simulink model "turbo_controller"  (R2025a)
settings: Solver=FixedStepAuto  StartTime=0.0  StopTime=inf  FixedStep=0.001  RelTol=1e-3
PostLoadFcn:
  | % 自动定位同目录CubeMX文件；不需要外部初始化脚本。
  | codertarget.data.setParameterValue('turbo_controller','STM32CubeMX.ProjectFile',fullfile(fileparts(get_param('turbo_controller','FileName')),'turbo_f407.ioc'));
InitFcn:
  | % 中文说明：按原控制器字段与类型创建三组接口总线；控制参数已内嵌。
  | tc_names=["EValve_Cycle" "EValve_Open" "Eblast_Cycle" "Eblast_Open" "Motor_Cycle" "Motor_Open" "EValve_Enable" "Eblast_Enable" "Motor_Enable" "SWO_Firework" "SWO_BleedAir" "EngineState" "Flag_ECUReset_Clear" "Flag_ECUReset_Save" "Flag_Reset_Enable" "Accelerator" "Nc_dem" "Nc"]; tc_types=["uint16" "uint16" "uint16" "uint16" "uint16" "uint16" "uint8" "uint8" "uint8" "uint8" "uint8" "uint8" "uint8" "uint8" "uint8" "single" "single" "single"];
  | for tc_k=1:numel(tc_names)
  |  tc_e(tc_k)=Simulink.BusElement; tc_e(tc_k).Name=char(tc_names(tc_k)); tc_e(tc_k).DataType=char(tc_types(tc_k));
  | end
  | EngineControl_Out=Simulink.Bus; EngineControl_Out.DataScope='Exported'; EngineControl_Out.Elements=tc_e;
  | clear tc_e tc_names tc_types tc_k
  | tc_names=["savedata1" "savedata2" "savedata3" "savedata4" "savedata5" "savedata6" "savedata7" "savedata8" "savedata9" "savedata10" "savedata11" "savedata12" "savedata13" "savedata14" "savedata15" "savedata16" "savedata17" "savedata18" "savedata19" "savedata20" "savedata21" "savedata22" "savedata23" "savedata24" "savedata25"]; tc_types=["single" "single" "single" "single" "single" "single" "single" "single" "single" "single" "single" "single" "single" "single" "single" "single" "single" "single" "single" "single" "single" "single" "single" "single" "single"];
  | for tc_k=1:numel(tc_names)
  |  tc_e(tc_k)=Simulink.BusElement; tc_e(tc_k).Name=char(tc_names(tc_k)); tc_e(tc_k).DataType=char(tc_types(tc_k));
  | end
  | SaveData_Out=Simulink.Bus; SaveData_Out.DataScope='Exported'; SaveData_Out.Elements=tc_e;
  | clear tc_e tc_names tc_types tc_k
  | tc_names=["senddata1" "senddata2" "senddata3" "senddata4" "senddata5" "senddata6" "senddata7" "senddata8" "senddata9" "senddata10" "senddata11" "senddata12" "senddata13" "senddata14" "senddata15" "senddata16" "senddata17" "senddata18" "senddata19" "senddata20" "senddata21" "senddata22" "senddata23" "senddata24" "senddata25" "senddata26" "senddata27" "senddata28" "senddata29"]; tc_types=["uint8" "uint8" "uint8" "uint8" "uint8" "uint8" "uint8" "uint8" "uint8" "uint8" "uint8" "uint8" "uint8" "uint8" "uint8" "uint8" "uint8" "uint8" "uint8" "uint8" "uint8" "uint8" "uint8" "uint8" "uint8" "uint8" "uint8" "uint8" "uint8"];
  | for tc_k=1:numel(tc_names)
  |  tc_e(tc_k)=Simulink.BusElement; tc_e(tc_k).Name=char(tc_names(tc_k)); tc_e(tc_k).DataType=char(tc_types(tc_k));
  | end
  | SendData_Out=Simulink.Bus; SendData_Out.DataScope='Exported'; SendData_Out.Elements=tc_e;
  | clear tc_e tc_names tc_types tc_k
  | 
  | % 以下为接口中文说明；只设置描述，不改变数值或数据类型。
  | EngineControl_Out.Description='执行控制输出（阀、电机、点火、状态及复位请求）';
  | tc_cn=["EValve_Cycle（主油阀周期计数（每计数2毫秒））" "EValve_Open（主油阀开通计数（每计数2毫秒））" "Eblast_Cycle（副油阀周期计数（每计数2毫秒））" "Eblast_Open（副油阀开通计数（每计数2毫秒））" "Motor_Cycle（起动电机周期计数）" "Motor_Open（起动电机开通计数）" "EValve_Enable（主油阀驱动使能）" "Eblast_Enable（副油阀驱动使能）" "Motor_Enable（起动电机使能）" "SWO_Firework（点火器使能（1开））" "SWO_BleedAir（引气阀使能（1开））" "EngineState（发动机状态）" "Flag_ECUReset_Clear（清除复位恢复状态请求）" "Flag_ECUReset_Save（保存复位恢复数据请求）" "Flag_Reset_Enable（处理器软件复位请求）" "Accelerator（油门／油泵给定控制量）" "Nc_dem（控制目标转速）" "Nc（发动机反馈转速（转每分））"];
  | tc_elements=EngineControl_Out.Elements;
  | for tc_k=1:numel(tc_cn)
  |  tc_elements(tc_k).Description=char(tc_cn(tc_k));
  | end
  | EngineControl_Out.Elements=tc_elements;
  | clear tc_cn tc_elements tc_k
  | SaveData_Out.Description='25项运行记录；字段含义按当前模型数据来源解释';
  | tc_cn=["savedata1（指令回显记录）" "savedata2（入口总温记录（℃））" "savedata3（电源电压记录）" "savedata4（排气温度记录（℃））" "savedata5（标定燃油压力记录）" "savedata6（副油阀占空比记录（％））" "savedata7（主油阀占空比记录（％））" "savedata8（温度修正转速记录）" "savedata9（开关输出及反馈位域）" "savedata10（物理转速记录）" "savedata11（油泵目标给定原始值）" "savedata12（起动电机占空比记录（％））" "savedata13（发动机状态码记录）" "savedata14（故障告警位域记录）" "savedata15（模型记录帧序号）" "savedata16（处理器温度记录（℃））" "savedata17（装订转速记录（沿用旧电源字段名））" "savedata18（导航高度记录）" "savedata19（飞行空速记录）" "savedata20（主阀旧记录位（恒零保留））" "savedata21（第21项保留记录（恒零））" "savedata22（保留记录项22）" "savedata23（保留记录项23）" "savedata24（保留记录项24）" "savedata25（保留记录项25）"];
  | tc_elements=SaveData_Out.Elements;
  | for tc_k=1:numel(tc_cn)
  |  tc_elements(tc_k).Description=char(tc_cn(tc_k));
  | end
  | SaveData_Out.Elements=tc_elements;
  | clear tc_cn tc_elements tc_k
  | SendData_Out.Description='29字段回传及外设命令接口；板端上位机帧只取第3至27字段';
  | tc_cn=["senddata1（回传发送允许标志（不直接上线路））" "senddata2（回传载荷长度25字节）" "senddata3（回传指令回显字节）" "senddata4（总温编码字节（℃＋80））" "senddata5（电源电压编码字节）" "senddata6（排温编码高字节）" "senddata7（排温编码低字节）" "senddata8（燃油压力编码高字节）" "senddata9（燃油压力编码低字节）" "senddata10（副油阀占空比字节（％））" "senddata11（主油阀占空比字节（％））" "senddata12（修正转速编码高字节）" "senddata13（修正转速编码低字节）" "senddata14（驱动及反馈状态位域）" "senddata15（物理转速编码高字节）" "senddata16（物理转速编码低字节）" "senddata17（油泵目标给定高字节（串口二使用））" "senddata18（油泵目标给定低字节（串口二使用））" "senddata19（起动电机占空比命令（串口一使用））" "senddata20（发动机状态码字节）" "senddata21（故障告警位域字节）" "senddata22（帧序号占位（板端另行填写））" "senddata23（处理器温度编码（℃＋50））" "senddata24（控制目标转速编码高字节）" "senddata25（控制目标转速编码低字节）" "senddata26（占位字节（板端改填实测泵速高字节））" "senddata27（占位字节（板端改填实测泵速低字节））" "senddata28（装订转速高字节（本板未发送））" "senddata29（装订转速低字节（本板未发送））"];
  | tc_elements=SendData_Out.Elements;
  | for tc_k=1:numel(tc_cn)
  |  tc_elements(tc_k).Description=char(tc_cn(tc_k));
  | end
  | SendData_Out.Elements=tc_elements;
  | clear tc_cn tc_elements tc_k
  | 
  | 
  | % FRAM模块化事务：接口类型和上电初始状态，随模型保存，无外部初始化文件。
  | clear FM_elements
  | FM_elements(1)=Simulink.BusElement;FM_elements(1).Name='phase';FM_elements(1).DataType='uint8';FM_elements(1).Dimensions=[1 1];FM_elements(1).Description='phase（当前事务阶段）';
  | FM_elements(2)=Simulink.BusElement;FM_elements(2).Name='a';FM_elements(2).DataType='uint8';FM_elements(2).Dimensions=[64 1];FM_elements(2).Description='a（启动时缓存的首区64字节）';
  | FM_elements(3)=Simulink.BusElement;FM_elements(3).Name='active';FM_elements(3).DataType='uint16';FM_elements(3).Dimensions=[1 1];FM_elements(3).Description='active（当前有效记录区地址）';
  | FM_elements(4)=Simulink.BusElement;FM_elements(4).Name='generation';FM_elements(4).DataType='uint32';FM_elements(4).Dimensions=[1 1];FM_elements(4).Description='generation（当前有效记录代号）';
  | FM_elements(5)=Simulink.BusElement;FM_elements(5).Name='record';FM_elements(5).DataType='uint8';FM_elements(5).Dimensions=[64 1];FM_elements(5).Description='record（本次冻结的待写记录）';
  | FM_elements(6)=Simulink.BusElement;FM_elements(6).Name='addr';FM_elements(6).DataType='uint16';FM_elements(6).Dimensions=[1 1];FM_elements(6).Description='addr（本次备用写入地址）';
  | FM_elements(7)=Simulink.BusElement;FM_elements(7).Name='lastSave';FM_elements(7).DataType='single';FM_elements(7).Dimensions=[1 1];FM_elements(7).Description='lastSave（上次开始保存的秒数）';
  | FM_elements(8)=Simulink.BusElement;FM_elements(8).Name='lastState';FM_elements(8).DataType='uint8';FM_elements(8).Dimensions=[1 1];FM_elements(8).Description='lastState（上次保存时的发动机状态）';
  | FM_elements(9)=Simulink.BusElement;FM_elements(9).Name='boot';FM_elements(9).DataType='boolean';FM_elements(9).Dimensions=[1 1];FM_elements(9).Description='boot（启动记录是否允许恢复）';
  | FM_elements(10)=Simulink.BusElement;FM_elements(10).Name='consumed';FM_elements(10).DataType='boolean';FM_elements(10).Dimensions=[1 1];FM_elements(10).Description='consumed（本次启动恢复通知是否已发送）';
  | FM_elements(11)=Simulink.BusElement;FM_elements(11).Name='payload';FM_elements(11).DataType='uint8';FM_elements(11).Dimensions=[20 1];FM_elements(11).Description='payload（当前20字节恢复内容）';
  | FM_elements(12)=Simulink.BusElement;FM_elements(12).Name='failures';FM_elements(12).DataType='uint32';FM_elements(12).Dimensions=[1 1];FM_elements(12).Description='failures（累计写后验证失败次数）';
  | FM_State=Simulink.Bus;FM_State.Elements=FM_elements;
  | clear FM_elements
  | FM_elements(1)=Simulink.BusElement;FM_elements(1).Name='validA';FM_elements(1).DataType='boolean';FM_elements(1).Dimensions=[1 1];FM_elements(1).Description='validA（首区记录有效）';
  | FM_elements(2)=Simulink.BusElement;FM_elements(2).Name='validB';FM_elements(2).DataType='boolean';FM_elements(2).Dimensions=[1 1];FM_elements(2).Description='validB（本次读回记录有效）';
  | FM_elements(3)=Simulink.BusElement;FM_elements(3).Name='generationA';FM_elements(3).DataType='uint32';FM_elements(3).Dimensions=[1 1];FM_elements(3).Description='generationA（首区代号）';
  | FM_elements(4)=Simulink.BusElement;FM_elements(4).Name='generationB';FM_elements(4).DataType='uint32';FM_elements(4).Dimensions=[1 1];FM_elements(4).Description='generationB（本次读回代号）';
  | FM_elements(5)=Simulink.BusElement;FM_elements(5).Name='payloadA';FM_elements(5).DataType='uint8';FM_elements(5).Dimensions=[20 1];FM_elements(5).Description='payloadA（首区恢复内容）';
  | FM_elements(6)=Simulink.BusElement;FM_elements(6).Name='payloadB';FM_elements(6).DataType='uint8';FM_elements(6).Dimensions=[20 1];FM_elements(6).Description='payloadB（本次读回恢复内容）';
  | FM_elements(7)=Simulink.BusElement;FM_elements(7).Name='recordB';FM_elements(7).DataType='uint8';FM_elements(7).Dimensions=[64 1];FM_elements(7).Description='recordB（本次读回的64字节原始记录）';
  | FM_Checked=Simulink.Bus;FM_Checked.Elements=FM_elements;
  | clear FM_elements
  | FM_elements(1)=Simulink.BusElement;FM_elements(1).Name='valid';FM_elements(1).DataType='boolean';FM_elements(1).Dimensions=[1 1];FM_elements(1).Description='valid（存在可选的有效启动记录）';
  | FM_elements(2)=Simulink.BusElement;FM_elements(2).Name='active';FM_elements(2).DataType='uint16';FM_elements(2).Dimensions=[1 1];FM_elements(2).Description='active（选中的记录地址）';
  | FM_elements(3)=Simulink.BusElement;FM_elements(3).Name='generation';FM_elements(3).DataType='uint32';FM_elements(3).Dimensions=[1 1];FM_elements(3).Description='generation（选中的记录代号）';
  | FM_elements(4)=Simulink.BusElement;FM_elements(4).Name='payload';FM_elements(4).DataType='uint8';FM_elements(4).Dimensions=[20 1];FM_elements(4).Description='payload（选中的恢复内容）';
  | FM_elements(5)=Simulink.BusElement;FM_elements(5).Name='boot';FM_elements(5).DataType='boolean';FM_elements(5).Dimensions=[1 1];FM_elements(5).Description='boot（选中记录是否允许恢复通知）';
  | FM_Startup=Simulink.Bus;FM_Startup.Elements=FM_elements;
  | FM_InitialState=struct('phase',uint8(0),'a',zeros(64,1,'uint8'),'active',uint16(768),'generation',uint32(0),'record',zeros(64,1,'uint8'),'addr',uint16(512),'lastSave',single(-1),'lastState',uint8(0),'boot',false,'consumed',false,'payload',zeros(20,1,'uint8'),'failures',uint32(0));
  | clear FM_elements
  | 
  | 
  | 
  | 
  | % BoardOutput模块化内部输出接口，保存在模型中，不依赖外部初始化文件。
  | clear BO_elements
  | BO_elements(1)=Simulink.BusElement;BO_elements(1).Name='portE';BO_elements(1).DataType='boolean';BO_elements(1).Dimensions=[3 1];BO_elements(1).Description='portE（E口三路输出电平）';
  | BO_elements(2)=Simulink.BusElement;BO_elements(2).Name='portD';BO_elements(2).DataType='boolean';BO_elements(2).Dimensions=[3 1];BO_elements(2).Description='portD（D口三路输出电平）';
  | BO_elements(3)=Simulink.BusElement;BO_elements(3).Name='tx4';BO_elements(3).DataType='uint8';BO_elements(3).Dimensions=[30 1];BO_elements(3).Description='tx4（上位机回传帧）';
  | BO_elements(4)=Simulink.BusElement;BO_elements(4).Name='len4';BO_elements(4).DataType='uint16';BO_elements(4).Dimensions=1;BO_elements(4).Description='len4（回传发送长度）';
  | BO_elements(5)=Simulink.BusElement;BO_elements(5).Name='tx1';BO_elements(5).DataType='uint8';BO_elements(5).Dimensions=[9 1];BO_elements(5).Description='tx1（电机指令帧）';
  | BO_elements(6)=Simulink.BusElement;BO_elements(6).Name='len1';BO_elements(6).DataType='uint16';BO_elements(6).Dimensions=1;BO_elements(6).Description='len1（电机发送长度）';
  | BO_elements(7)=Simulink.BusElement;BO_elements(7).Name='tx2';BO_elements(7).DataType='uint8';BO_elements(7).Dimensions=[9 1];BO_elements(7).Description='tx2（油泵指令帧）';
  | BO_elements(8)=Simulink.BusElement;BO_elements(8).Name='len2';BO_elements(8).DataType='uint16';BO_elements(8).Dimensions=1;BO_elements(8).Description='len2（油泵发送长度）';
  | BO_Output=Simulink.Bus;BO_Output.Elements=BO_elements;clear BO_elements
model workspace (MAT data in the model file):
  CRC16_Table_Reference = [0; 4129; 8258; 12387; 16516; 20645; 24774; 28903; 33032; 37161; 41290; 45419; 49548; 53677; 57806; 61935; 4657; 528; 12915; 8786; 21173; 17044; 29431; 25302; 37689; 33560; 45947; 41818; 54205; 50076; 62463; 58334; 9314; 13379; 1056; 5121; 25830; 29895; 17572; 21637; 42346; 46411; 34088; 38153; 58862; 62927; 50604; 54669; 13907; 9842; 5649; 1584; 30423; 26358; 22165; 18100; 46939; 42874; 38681; 34616; 63455; 59390; 55197; 51132; 18628; 22757; 26758; 30887; 2112; 6241; 10242; 14371; 51660; 55789; 59790; 63919; 35144; 39273; 43274; 47403; 23285; 19156; 31415; 27286; 6769; 2640; 14899; 10770; 56317; 52188; 64447; 60318; 39801; 35672; 47931; 43802; 27814; 31879; 19684; 23749; 11298; 15363; 3168; 7233; 60846; 64911; 52716; 56781; 44330; 48395; 36200; 40265; 32407; 28342; 24277; 20212; 15891; 11826; 7761; 3696; 65439; 61374; 57309; 53244; 48923; 44858; 40793; 36728; 37256; 33193; 45514; 41451; 53516; 49453; 61774; 57711; 4224; 161; 12482; 8419; 20484; 16421; 28742; 24679; 33721; 37784; 41979; 46042; 49981; 54044; 58239; 62302; 689; 4752; 8947; 13010; 16949; 21012; 25207; 29270; 46570; 42443; 38312; 34185; 62830; 58703; 54572; 50445; 13538; 9411; 5280; 1153; 29798; 25671; 21540; 17413; 42971; 47098; 34713; 38840; 59231; 63358; 50973; 55100; 9939; 14066; 1681; 5808; 26199; 30326; 17941; 22068; 55628; 51565; 63758; 59695; 39368; 35305; 47498; 43435; 22596; 18533; 30726; 26663; 6336; 2273; 14466; 10403; 52093; 56156; 60223; 64286; 35833; 39896; 43963; 48026; 19061; 23124; 27191; 31254; 2801; 6864; 10931; 14994; 64814; 60687; 56684; 52557; 48554; 44427; 40424; 36297; 31782; 27655; 23652; 19525; 15522; 11395; 7392; 3265; 61215; 65342; 53085; 57212; 44955; 49082; 36825; 40952; 28183; 32310; 20053; 24180; 11923; 16050; 3793; 7920]
  PE_Kaer = [0.15402 0.15402 0.12264 0.10076 0.09481 0.07601 0.07111 0.0569 0.05198 0.04926 0.05308 0.04325 0.04325]
  PE_Nr = [21.2982 61.4260372 67.7475458 72.7394382 76.845934 80.6988798 83.8449282 86.6491912 88.9382406 89.178606 91.1938214 93.4068058 104.4626]
  PE_Pump_Translate = 33.5999984741
  PE_RotaSpeed_Translate = 860
  PE_Taer = [0.4939154 0.4939154 0.40780982 0.34066978 0.31622756 0.30405716 0.34300244 0.26785022 0.37393554 0.23914836 0.44563948 0.31044662 0.31044662]
  PF_ACCFULLRANGE = 3360
  PF_Flag_ECUReset = 0
  PF_Flag_rx_suc = 1
  PF_Gear_Info = [40000; 45000; 50000; 55000; 57000; 59000; 60000; 61000; 61000; 61000; 61000; 61000]
  PF_K_TiaoJie = 1
  PF_Kpu = 10
  PF_MySet_Rxdata = [0; 0; 0; 0; 0; 0; 0; 0; 0; 0; 0; 0; 0; 0; 0; 0; 0; 0; 0; 0; 0; 0; 0; 0; 0; 0; 0; 0; 0; 0; 0; 0; 0; 0; 0; 0; 0; 0; 0; 0; 0; 0; 0; 0; 0; 0; 0; 0; 0; 0]
  PF_MyUsart1_Rxdata = [0; 0; 0; 0; 0; 0; 0; 0; 0; 0; 0; 0; 0; 0; 0; 0; 0; 0; 0; 0; 0; 0; 0; 0; 0; 0; 0; 0; 0; 0; 0; 0; 0; 0; 0; 0; 0; 0; 0; 0; 0; 0; 0; 0; 0; 0; 0; 0; 0; 0]
  PF_MyUsart2_Rxdata = [0; 0; 0; 0; 0; 0; 0; 0; 0; 0; 0; 0; 0; 0; 0; 0; 0; 0; 0; 0; 0; 0; 0; 0; 0; 0; 0; 0; 0; 0; 0; 0; 0; 0; 0; 0; 0; 0; 0; 0; 0; 0; 0; 0; 0; 0; 0; 0; 0; 0]
  PF_Reset_Information = [0; 0; 0; 0; 0; 0; 0; 0; 0; 0; 0; 0; 0; 0; 0; 0; 0; 0; 0; 0]
  PF_Sensor_X1_T4 = [0 4095]
  PF_Sensor_X2_T4 = [0 1.66666698456]
  PF_Sensor_X3_T4 = [0 504 999 1497 2010 2529 3051 3568 4076 4571 4959]
  PF_Sensor_X_P2 = [0.5 3]
  PF_Sensor_X_Poil = [0.5 3]
  PF_Sensor_X_T1t = [-50 300]
  PF_Sensor_X_Vpower = [0 3]
  PF_Sensor_X_Vpump = [0 3]
  PF_Sensor_Y1_T4 = [0 3]
  PF_Sensor_Y2_T4 = [0 5000]
  PF_Sensor_Y3_T4 = [0 100 200 300 400 500 600 700 800 900 980]
  PF_Sensor_Y_P2 = [0 1000]
  PF_Sensor_Y_Poil = [0 1000]
  PF_Sensor_Y_T1t = [-50 300]
  PF_Sensor_Y_Vpower = [0 33]
  PF_Sensor_Y_Vpump = [0 33]
  PG_CtrlMode_CloseLoop = mpt.Parameter
  PG_CtrlMode_CloseLoop.Value = 2
  PG_CtrlMode_CloseLoop.Complexity = 'real'
  PG_CtrlMode_CloseLoop.Dimensions = [1 1]
  PG_CtrlMode_CloseLoop.DataType = 'uint8'
  PG_CtrlMode_ManualAcc = mpt.Parameter
  PG_CtrlMode_ManualAcc.Value = 3
  PG_CtrlMode_ManualAcc.Complexity = 'real'
  PG_CtrlMode_ManualAcc.Dimensions = [1 1]
  PG_CtrlMode_ManualAcc.DataType = 'uint8'
  PG_CtrlMode_Origin = mpt.Parameter
  PG_CtrlMode_Origin.Value = 0
  PG_CtrlMode_Origin.Complexity = 'real'
  PG_CtrlMode_Origin.Dimensions = [1 1]
  PG_CtrlMode_Origin.DataType = 'uint8'
  PG_CtrlMode_Start = mpt.Parameter
  PG_CtrlMode_Start.Value = 1
  PG_CtrlMode_Start.Complexity = 'real'
  PG_CtrlMode_Start.Dimensions = [1 1]
  PG_CtrlMode_Start.DataType = 'uint8'
  PG_CtrlMode_Stop = mpt.Parameter
  PG_CtrlMode_Stop.Value = 4
  PG_CtrlMode_Stop.Complexity = 'real'
  PG_CtrlMode_Stop.Dimensions = [1 1]
  PG_CtrlMode_Stop.DataType = 'uint8'
  PG_ES_Clp = mpt.Parameter
  PG_ES_Clp.Value = 2
  PG_ES_Clp.Complexity = 'real'
  PG_ES_Clp.Dimensions = [1 1]
  PG_ES_Clp.DataType = 'uint8'
  PG_ES_EngStart = mpt.Parameter
  PG_ES_EngStart.Value = 1
  PG_ES_EngStart.Complexity = 'real'
  PG_ES_EngStart.Dimensions = [1 1]
  PG_ES_EngStart.DataType = 'uint8'
  PG_ES_Manual = mpt.Parameter
  PG_ES_Manual.Value = 3
  PG_ES_Manual.Complexity = 'real'
  PG_ES_Manual.Dimensions = [1 1]
  PG_ES_Manual.DataType = 'uint8'
  PG_ES_Origin = mpt.Parameter
  PG_ES_Origin.Value = 0
  PG_ES_Origin.Complexity = 'real'
  PG_ES_Origin.Dimensions = [1 1]
  PG_ES_Origin.DataType = 'uint8'
  PG_ES_Stop = mpt.Parameter
  PG_ES_Stop.Value = 4
  PG_ES_Stop.Complexity = 'real'
  PG_ES_Stop.Dimensions = [1 1]
  PG_ES_Stop.DataType = 'uint8'
  PG_Instr_BleedAirSet = mpt.Parameter
  PG_Instr_BleedAirSet.Value = 14
  PG_Instr_BleedAirSet.Complexity = 'real'
  PG_Instr_BleedAirSet.Dimensions = [1 1]
  PG_Instr_BleedAirSet.DataType = 'uint8'
  PG_Instr_CloseLoop = mpt.Parameter
  PG_Instr_CloseLoop.Value = 3
  PG_Instr_CloseLoop.Complexity = 'real'
  PG_Instr_CloseLoop.Dimensions = [1 1]
  PG_Instr_CloseLoop.DataType = 'uint8'
  PG_Instr_ECUReSet = mpt.Parameter
  PG_Instr_ECUReSet.Value = 9
  PG_Instr_ECUReSet.Complexity = 'real'
  PG_Instr_ECUReSet.Dimensions = [1 1]
  PG_Instr_ECUReSet.DataType = 'uint8'
  PG_Instr_EValveSet = mpt.Parameter
  PG_Instr_EValveSet.Value = 11
  PG_Instr_EValveSet.Complexity = 'real'
  PG_Instr_EValveSet.Dimensions = [1 1]
  PG_Instr_EValveSet.DataType = 'uint8'
  PG_Instr_EblastSet = mpt.Parameter
  PG_Instr_EblastSet.Value = 12
  PG_Instr_EblastSet.Complexity = 'real'
  PG_Instr_EblastSet.Dimensions = [1 1]
  PG_Instr_EblastSet.DataType = 'uint8'
  PG_Instr_Erase = mpt.Parameter
  PG_Instr_Erase.Value = 0
  PG_Instr_Erase.Complexity = 'real'
  PG_Instr_Erase.Dimensions = [1 1]
  PG_Instr_Erase.DataType = 'uint8'
  PG_Instr_FireWorkSet = mpt.Parameter
  PG_Instr_FireWorkSet.Value = 10
  PG_Instr_FireWorkSet.Complexity = 'real'
  PG_Instr_FireWorkSet.Dimensions = [1 1]
  PG_Instr_FireWorkSet.DataType = 'uint8'
  PG_Instr_ManualPlus = mpt.Parameter
  PG_Instr_ManualPlus.Value = 4
  PG_Instr_ManualPlus.Complexity = 'real'
  PG_Instr_ManualPlus.Dimensions = [1 1]
  PG_Instr_ManualPlus.DataType = 'uint8'
  PG_Instr_ManualrReduce = mpt.Parameter
  PG_Instr_ManualrReduce.Value = 5
  PG_Instr_ManualrReduce.Complexity = 'real'
  PG_Instr_ManualrReduce.Dimensions = [1 1]
  PG_Instr_ManualrReduce.DataType = 'uint8'
  PG_Instr_MotorSet = mpt.Parameter
  PG_Instr_MotorSet.Value = 13
  PG_Instr_MotorSet.Complexity = 'real'
  PG_Instr_MotorSet.Dimensions = [1 1]
  PG_Instr_MotorSet.DataType = 'uint8'
  PG_Instr_OilSet = mpt.Parameter
  PG_Instr_OilSet.Value = 8
  PG_Instr_OilSet.Complexity = 'real'
  PG_Instr_OilSet.Dimensions = [1 1]
  PG_Instr_OilSet.DataType = 'uint8'
  PG_Instr_SelfCheck = mpt.Parameter
  PG_Instr_SelfCheck.Value = 7
  PG_Instr_SelfCheck.Complexity = 'real'
  PG_Instr_SelfCheck.Dimensions = [1 1]
  PG_Instr_SelfCheck.DataType = 'uint8'
  PG_Instr_Start = mpt.Parameter
  PG_Instr_Start.Value = 1
  PG_Instr_Start.Complexity = 'real'
  PG_Instr_Start.Dimensions = [1 1]
  PG_Instr_Start.DataType = 'uint8'
  PG_Instr_Stop = mpt.Parameter
  PG_Instr_Stop.Value = 6
  PG_Instr_Stop.Complexity = 'real'
  PG_Instr_Stop.Dimensions = [1 1]
  PG_Instr_Stop.DataType = 'uint8'
  PG_Instr_StopZero = Simulink.Parameter
  PG_Instr_StopZero.Value = 15
  PG_Instr_StopZero.Complexity = 'real'
  PG_Instr_StopZero.Dimensions = [1 1]
  PG_Instr_StopZero.DataType = 'uint8'
  PG_Location_Air = Simulink.Parameter
  PG_Location_Air.Value = 2
  PG_Location_Air.Complexity = 'real'
  PG_Location_Air.Dimensions = [1 1]
  PG_Location_Air.DataType = 'uint8'
  PG_Location_Gnd = Simulink.Parameter
  PG_Location_Gnd.Value = 1
  PG_Location_Gnd.Complexity = 'real'
  PG_Location_Gnd.Dimensions = [1 1]
  PG_Location_Gnd.DataType = 'uint8'
  PG_ServoCtrlMode_CloseLoop = Simulink.Parameter
  PG_ServoCtrlMode_CloseLoop.Value = 31
  PG_ServoCtrlMode_CloseLoop.Complexity = 'real'
  PG_ServoCtrlMode_CloseLoop.Dimensions = [1 1]
  PG_ServoCtrlMode_CloseLoop.DataType = 'uint8'
  PG_ServoCtrlMode_CloseLoopMax = Simulink.Parameter
  PG_ServoCtrlMode_CloseLoopMax.Value = 32
  PG_ServoCtrlMode_CloseLoopMax.Complexity = 'real'
  PG_ServoCtrlMode_CloseLoopMax.Dimensions = [1 1]
  PG_ServoCtrlMode_CloseLoopMax.DataType = 'uint8'
  PG_ServoCtrlMode_CloseLoopMin = Simulink.Parameter
  PG_ServoCtrlMode_CloseLoopMin.Value = 33
  PG_ServoCtrlMode_CloseLoopMin.Complexity = 'real'
  PG_ServoCtrlMode_CloseLoopMin.Dimensions = [1 1]
  PG_ServoCtrlMode_CloseLoopMin.DataType = 'uint8'
  PG_ServoCtrlMode_ManualAcc = Simulink.Parameter
  PG_ServoCtrlMode_ManualAcc.Value = 21
  PG_ServoCtrlMode_ManualAcc.Complexity = 'real'
  PG_ServoCtrlMode_ManualAcc.Dimensions = [1 1]
  PG_ServoCtrlMode_ManualAcc.DataType = 'uint8'
  PG_ServoCtrlMode_ManualAccMax = Simulink.Parameter
  PG_ServoCtrlMode_ManualAccMax.Value = 22
  PG_ServoCtrlMode_ManualAccMax.Complexity = 'real'
  PG_ServoCtrlMode_ManualAccMax.Dimensions = [1 1]
  PG_ServoCtrlMode_ManualAccMax.DataType = 'uint8'
  PG_ServoCtrlMode_ManualAccMin = Simulink.Parameter
  PG_ServoCtrlMode_ManualAccMin.Value = 23
  PG_ServoCtrlMode_ManualAccMin.Complexity = 'real'
  PG_ServoCtrlMode_ManualAccMin.Dimensions = [1 1]
  PG_ServoCtrlMode_ManualAccMin.DataType = 'uint8'
  PG_SpeedDot_Permit = Simulink.Parameter
  PG_SpeedDot_Permit.Value = 4000
  PG_SpeedDot_Permit.Complexity = 'real'
  PG_SpeedDot_Permit.Dimensions = [1 1]
  PG_SpeedDot_Permit.DataType = 'single'
  PL_EngineModel_Actuator = [0 10 100]
  PL_EngineModel_EngineStar_Press_P2 = [1013 1098.4 1099.144828 1099.931034 1103.613793 1162.662069 1143.793103 1131.006897 1123.186207 1117.6 1114 1111.806897 1110.524138 1109.82069 1109.655172 1109.82069 1110.151724 1110.689655 1111.475862 1112.344828 1113.337931 1114.496552 1115.655172 1116.896552 1118.137931 1119.503448 1120.910345 1122.275862 1123.682759 1125.255172 1126.910345 1128.524138 1130.055172 1131.627586 1133.241379 1134.937931 1136.675862 1138.496552 1140.193103 1142.8 1143.917241 1145.737931 1147.682759 1149.42069 1151.448276 1153.393103 1155.296552 1157.282759 1159.393103 1161.503448 1163.489655 1165.517241 1167.544828 1169.655172 1171.806897 1173.958621 1176.275862 1178.551724 1180.868966 1183.393103 1185.793103 1188.068966 1190.427586 1192.703448 1195.351724 1197.793103 1199.986207 1202.427586 1204.827586 1207.227586 1209.958621 1212.524138 1215.172414 1217.903448 1220.8 1223.448276 1229.613793 1231.558621 1233.462069 1236.855172 1238.717241 1241.903448 1245.255172 1248.689655 1252.248276 1255.682759 1259.531034 1263.255172 1267.393103 1271.406897 1275.875862 1280.055172 1284.068966 1288.827586 1293.048276 1297.972414 1302.813793 1307.531034 1312.496552 1317.586207 1322.8 1328.758621 1334.882759 1340.841379 1347.048276 1353.710345 1360 1367.696552 1374.524138 1380.97931 1388.593103 1396.703448 1405.682759 1414.455172 1423.972414 1433.696552 1444.537931 1455.834483 1468.165517 1486.413793 1494.068966 1507.434483 1521.958621 1536.813793 1553.613793 1570.786207 1589.448276]
  PL_EngineModel_EngineStar_RotaSpeed = [200 2000 9584 9660 10220 10240 10260 10288 10308 10368 10380 10408 10484 10596 10600 10616 10648 10700 10776 10860 10956 11068 11180 11300 11420 11552 11688 11820 11956 12108 12268 12424 12572 12724 12880 13044 13212 13388 13552 13804 13912 14088 14276 14444 14640 14828 15012 15204 15408 15612 15804 16000 16196 16400 16608 16816 17040 17260 17484 17728 17960 18180 18408 18628 18884 19120 19332 19568 19800 20032 20296 20544 20800 21064 21344 21600 22196 22384 22568 22896 23076 23384 23708 24040 24384 24716 25088 25448 25848 26236 26668 27072 27460 27920 28328 28804 29272 29728 30208 30700 31204 31780 32372 32948 33548 34192 34800 35544 36204 36828 37564 38348 39216 40064 40984 41924 42972 44064 45256 47020 47760 49052 50456 51892 53516 55176 56980]
  PL_EngineModel_EngineStar_Temp_Exhaust = [128 129 129.1 130 131 131.1 132 133 134 134.1 135 135.1 136 136.1 137 137.1 138 139 139.1 140 141 143 144 146 148 149 151 154 156 160 164 168 173 178 183 188 194 200 207 214 218 224 231 237 243 250 256 263 269 276 282 289 295 302 309 316 323 329 334 339 344 348 351 354 357 360 362 365 368 370 373 375 378 380 382 384 387 389 392 395 396 400 403 406 409 412 415 418 421 425 429 433 437 441 445 448 452 456 460 464 468 472 477 482 487 493 500 507 513 519 526 532 539 547 557 568 580 593 607 623 632 648 663 677 690 702 712]
  PL_EngineModel_EngineStar_Time = [0.05 0.1 0.15 0.2 0.25 0.3 0.35 0.4 0.45 0.5 0.55 0.6 0.65 0.7 0.75 0.8 0.85 0.9 0.95 1 1.05 1.1 1.15 1.2 1.25 1.3 1.35 1.4 1.45 1.5 1.55 1.6 1.65 1.7 1.75 1.8 1.85 1.9 1.95 2 2.05 2.1 2.15 2.2 2.25 2.3 2.35 2.4 2.45 2.5 2.55 2.6 2.65 2.7 2.75 2.8 2.85 2.9 2.95 3 3.05 3.1 3.15 3.2 3.25 3.3 3.35 3.4 3.45 3.5 3.55 3.6 3.65 3.7 3.75 3.8 3.85 3.9 3.95 4 4.05 4.1 4.15 4.2 4.25 4.3 4.35 4.4 4.45 4.5 4.55 4.6 4.65 4.7 4.75 4.8 4.85 4.9 4.95 5 5.05 5.1 5.15 5.2 5.25 5.3 5.35 5.4 5.45 5.5 5.55 5.6 5.65 5.7 5.75 5.8 5.85 5.9 5.95 6 6.05 6.1 6.15 6.2 6.25 6.3 6.35]
  PL_EngineModel_IdleAbove_Nr = [0 21.2982 61.4260372 67.7475458 72.7394382 76.845934 80.6988798 83.8449282 86.6491912 88.9382406 89.178606 91.1938214 93.4068058 104.4626]
  PL_EngineModel_IdleAbove_P2r = [0.986923266716 1.57907722675 1.81593881076 1.99358499877 2.23044658278 2.43770046879 2.65482358747 2.84233900814 3.03972366149 3.18776215149 3.25684678016 3.3950160375 3.50357759684 4.04638539354]
  PL_EngineModel_IdleAbove_Tempr = [0.0536001429337 1.07200285867 1.63301768805 1.63659103091 1.66875111667 1.72592460247 1.77595140254 1.86171163123 1.95461854565 2.03323208862 2.03323208862 2.13685903162 2.24405931749 2.57280686082]
  PL_EngineModel_IdleAbove_Ter = [0.42434128 0.42434128 0.42434128 0.30669408 0.23570008 0.22150128 0.1997974 0.23803274 0.16115638 0.24279948 0.13600422 0.31308354 0.1937122 0.1937122]
  PL_EngineModel_IdleAbove_Wfr = [0 10.142 23.8337 27.8905 31.9473 36.0041 40.0609 44.1177 48.1745 52.2313 52.7384 56.7952 60.852 81.136]
  PL_EngineModel_Press_P2 = [400 400 400 400 400 400 400 400 400 400]
  PL_EngineModel_Rotaspeed = [0 20000 96400]
  PL_EngineModel_Temp_Exhaust = [500 500 500 500 500 500 500 500 500 500]
  PL_Kaer = [0.1 0.1 0.1 0.1 0.1 0.1]
  PL_Nr = [50 60 70 80 90 100]
  PL_Taer = [0.1 0.1 0.1 0.1 0.1 0.1]
  Sig = Simulink.Signal
  Sig.Dimensions = -1
  Sig.DimensionsMode = 'auto'
  Sig.Complexity = 'auto'
  Sig.SampleTime = -1
  Sig.SamplingMode = 'auto'
  Sig.DataType = 'auto'
  Ts_ms = Simulink.Parameter
  Ts_ms.Value = 20
  Ts_ms.Complexity = 'real'
  Ts_ms.Dimensions = [1 1]
  Ts_ms.DataType = 'single'
  false = Simulink.Parameter
  false.Value = 0
  false.Complexity = 'real'
  false.Dimensions = [1 1]
  false.DataType = 'boolean'
  true = Simulink.Parameter
  true.Value = 1
  true.Complexity = 'real'
  true.Dimensions = [1 1]
  true.DataType = 'boolean'
libraries: simulink x97, stm32blockslib x10, stm32f4xxblockslib x8
(part 1 of 26)
Description:
  | 维护文件只有 turbo_controller.slx 与 turbo_f407.ioc；无独立手写C文件、驱动、任务或初始化脚本。
  | 一、职责：CubeMX配置引脚、时钟、ADC、DMA、UART、SPI、定时捕获、SDIO、FatFs与FreeRTOS。官方STM32支持包模块访问外设。原控制核心CLM、ESM、FPM、MAM、SDM等保留在模型中，固定20ms执行；BoardInput、BoardOutput、FramRecovery实现协议、换算、驱动时序与恢复事务，均由模型生成。
  | 二、板级：STM32F407VGT6，8MHz外部晶振，168MHz主频。UART4上位机，USART1起动电机，USART2油泵，均115200；SPI2模式3连接FRAM。保留原执行器和反馈引脚。
  | 三、记录：官方SD卡MAT文件记录，SDIO四位总线，FatFs长文件名。engine_log每20ms一行：第1至25列对应savedata1至savedata25，第26列为模型时间秒，第27列为FRAM写入错误计数。读取SD卡MAT文件后可用MATLAB自带工具查看/导出，无自定义解码文件。
  | 重要待确认：原板未找到独立卡检测接线。PC0仅作为SD_DETECT_PENDING配置占位，低电平表示插卡，未确认实板可用，不代表原板已经连接该信号。请按实际原理图确认或更换此输入；在确认前不能认为SD记录可直接运行。原PE12等反馈引脚不作为卡检测。
  | 四、恢复：FRAM使用0x0200/0x0300两个64字节副本、代次号、CRC32、最后提交标记；不覆盖或读取旧0x0000/0x0100槽。有效启动/运行记录可在模型中恢复。油门高低字节正确分开，修正旧代码重复取高字节的问题。
  | 五、迁移差异：油压按当前模型接口输入原始ADC码，旧板代码曾传入已换算电压，需压力源标定核验。转速捕获使用1MHz计数、3脉冲每转、去极值滤波与100ms无边沿判零，低速与抖动需实板比较。点火在模型内实现9ms开/1ms关；主副阀按2ms计数。A55A参数装订扩展沿用旧工程零配置输入，未新增其协议。未新增旧工程中已注释的看门狗策略。
  | 六、验证：整模型更新、类型推导已通过；根层连线检查通过。未烧录、未实板试车，完整ARM编译尚未完成。配置工具拒绝同时保留STM32F4官方硬件板绑定和直接芯片设置；没有为绕过此限制清除官方板绑定。本文件不应被当作已验收可烧录工程。
  | 七、版本：MATLAB R2025a Update1，STM32官方支持包25.1.0，CubeMX6.12.0，STM32CubeF4 1.28.0。首次构建需上述官方依赖；CubeMX与Simulink将自动生成目录及源码，这些是构建产物，不是额外维护源文件。生成代码受本机学术许可证限制。
  | 打开本模型后，硬件配置自动定位同目录turbo_f407.ioc；无需外部路径初始化脚本。
settings Model: STM32="{\"AnalogInput\":{\"ID\":\"turbo_controller:535549\"},\"DigitalPortRead\":[{\"ID\":\"turbo_controller:535550\"},{\"ID\":\"turbo_controller:535551\"},{\"ID\":\"turbo_controller:538340\"},{\"ID\":\"turbo_controller:538341\"},{\"ID\":\"turbo_controller:538342\"}],\"TimerCapture\":{\"ID\":\"turbo_controller:535552\"},\"UARTRead\":[{\"ID\":\"turbo_controller:535560\"},{\"ID\":\"turbo_controller:535562\"},{\"ID\":\"turbo_controller:535564\"}],\"UARTWrite\":[{\"ID\":\"turbo_controller:535561\"},{\"ID\":\"turbo_controller:535563\"},{\"ID\":\"turbo_controller:535565\"}],\"DigitalPortWrite\":[{\"ID\":\"turbo_controller:535568\"},{\"ID\":\"turbo_controller:535569\"}],\"SPIControllerTransfer\":[{\"ID\":\"turbo_controller:535599\"},{\"ID\":\"turbo_controller:535600\"},{\"ID\":\"turbo_controller:535601\"}]}"  TunableVars=PF_ACCFULLRANGE,PF_Gear_Info,PF_ManualAcc_Info,PF_MyUsart2_Rxdata,PF_SpeedSet_Info,PF_Speed_Info,PF_Start_Info  TunableVarsStorageClass=Auto,Auto,Auto,Auto,Auto,Auto,Auto  TunableVarsTypeQualifier=,,,,,,  Creator=wubin  LastModifiedBy=ZHOU JIANHUA
settings SolverCC: AlgebraicLoopSolver=TrustRegion
settings DataIOCC: LimitDataPoints=on  SaveOutput=off  SignalLogging=off  SaveTime=off  ReturnWorkspaceOutputs=off
settings OptimizationCC: DefaultParameterBehavior=Inlined  UseDivisionForNetSlopeComputation=on  GainParamInheritBuiltInType=on  UseFloatMulNetSlope=on  InlineInvariantSignals=on  PassReuseOutputArgsAs=Individual arguments  NoFixptDivByZeroProtection=on  EfficientFloat2IntCast=on  LifeSpan=1  MaxStackSize=64  EfficientTunableParamExpr=on
settings DebuggingCC: UnconnectedInputMsg=warning  UnconnectedOutputMsg=warning  UnconnectedLineMsg=warning  AllowSymbolicDim=off  SFUnexpectedBacktrackingDiag=warning  SFNoUnconditionalDefaultTransitionDiag=warning  SFExecutionAtInitializationDiag=none  ArithmeticOperatorsInVariantConditions=warning
settings HardwareCC: ProdBitPerPointer=32.0  ProdBitPerSizeT=32.0  ProdBitPerPtrDiffT=32.0  ProdLargestAtomicInteger=Long  ProdLargestAtomicFloat=Double  ProdWordSize=32.0  ProdLongLongMode=on  ProdHWDeviceType=ARM Compatible->ARM Cortex-M
settings ModelReferenceCC: EnableRefExpFcnMdlSchedulingChecks=on  PropagateSignalLabelsOutOfModel=off
settings SFSimCC: SimCustomHeaderCode=void NVIC_SystemReset(void);  SimUseLocalCustomCode=off  MATLABDynamicMemAlloc=off  CustomCodeUndefinedFunction=UseInterfaceOnly
settings RTWCC: SystemTargetFile=ert.tlc  HardwareBoard=STM32F4xx Based  TLCOptions="-aInlineSetEventsForThisBaseRateFcn=TLC_FALSE -aSuppressMultiTaskScheduler=TLC_FALSE  -aRateBasedStepFcn=0"  TemplateMakefile=ert_default_tmf  GenerateReport=on  RTWUseLocalCustomCode=off  CustomHeaderCode="#include \"stm32f4xx.h\""  Toolchain=Armclang Compiler  IncludeHyperlinkInReport=on  PortableWordSizes=on  CreateSILPILBlock=SIL  GenerateTraceInfo=on  GenerateTraceReport=on  GenerateTraceReportSl=on  GenerateTraceReportSf=on  GenerateTraceReportEml=on  GenerateCodeMetricsReport=on  GPUComputeCapability=3.5  Description=Embedded Coder
settings CodeAppCC: ForceParamTrailComments=on  IgnoreCustomStorageClasses=off  SimulinkDataObjDesc=on  CustomSymbolStrGlobalVar=rt$N$M  CustomSymbolStrType=$N$M  CustomSymbolStrFcn=$N$M$F  CustomSymbolStrMacro=$N$M  InsertBlockDesc=on
settings ERTTargetCC: ExtModeTransport=3.0  ExtModeStaticAllocSize=2048.0  RootIOFormat=Structure reference  ConvertIfToSwitch=off  SuppressUnreachableDefaultCases=off  EnableUserReplacementTypes=on  DynamicArrayContainerType=coder::array  TargetLangStandard=C99 (ISO)  CodeReplacementLibrary=ARM Cortex-M  MultiwordLength=2048.0  IncludeMdlTerminateFcn=off  CombineSignalStateStructs=on  MatFileLogging=on  SupportContinuousTime=on  SupportNonInlinedSFcns=on  SupportVariableSizeSignals=on
settings ConfigComp: CovMetricSettings=dw  CovSaveCumulativeToWorkspaceVar=on  CovSaveSingleToWorkspaceVar=on  CovExternalEMLEnable=off

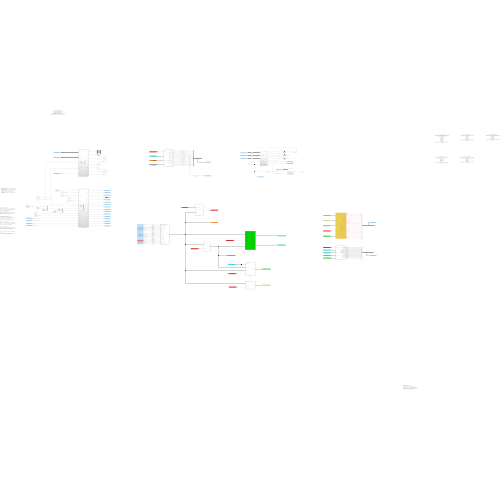
[thumbnail: Simulink's stored preview of the top-level diagram]
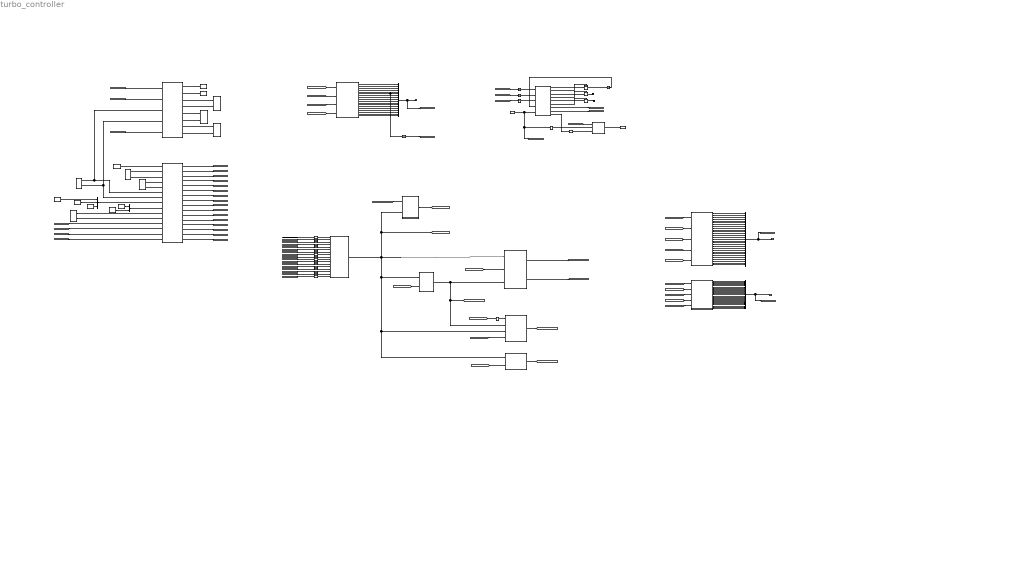
== system turbo_controller ==
  note: 【本页库子系统中文说明】ADC1_八路采样
      | 一、它做什么？
      | 这是MathWorks官方ADC采样块，从CubeMX配置的ADC读取模拟输入。当前配置8路转换，
      | 采样时间0.02秒（20毫秒）；后续BoardInput每1毫秒处理时可能多次使用最近一次采
      | 样值，不代表ADC每毫秒都重新测量。读到的是原始计数，工程量的比例、标定和滤波
      | 在后面的模型中完成。引脚和外设初始化以CubeMX配置为准。
      | 二、本实例当前参数
      | ADC外设：ADC1
      | 转换组：常规转换组
      | 触发与读取模式：触发并读取
      | 转换通道数：8
      | 是否启用转换缓冲：关闭
      | 缓冲长度：1
      | 是否输出状态：关闭
      | 采样时间（秒）：0.02
      | 是否启用仿真输入：关闭
      | 三、怎样继续学习？
      | 这是标准库子系统实例。中文说明放在使用它的父级页面，并同步存入本块Descriptio
      | n（模块说明）；官方库链接保留。先看本实例的输入来自哪里、输出交给谁，再结合
      | 以上参数理解作用。
  note: 【本页库子系统中文说明】GPIOD_两路报警
      | 一、它做什么？
      | 这是官方数字端口读取块，读取指定GPIO端口/引脚当前的高低电平，再交给输入映射
      | 模块解释为反馈或告警。高电平不必然代表“正常”或“开启”，要结合电路极性和后
      | 面的取反逻辑。它只读反馈，不在这里产生输出驱动。
      | 二、本实例当前参数
      | 端口名称：GPIOD
      | PinNumber：[8 9]
      | ReadOperation：开启
      | IOAsArray：开启
      | 采样时间（秒）：0.001
      | 是否启用仿真输入：关闭
      | 三、怎样继续学习？
      | 这是标准库子系统实例。中文说明放在使用它的父级页面，并同步存入本块Descriptio
      | n（模块说明）；官方库链接保留。先看本实例的输入来自哪里、输出交给谁，再结合
      | 以上参数理解作用。
  note: 【本页库子系统中文说明】GPIOD_使能镜像点火
      | 一、它做什么？
      | 这是官方数字端口写入块，把模型传来的高低电平写到已配置的GPIO端口。前面的Boar
      | dOutput已处理周期、使能和电平极性，这里负责真正交给硬件；板级引脚初始化由Cub
      | eMX生成。软件值与阀门的通断关系取决于外部电路，不应仅凭0或1猜动作。
      | 二、本实例当前参数
      | 端口名称：GPIOD
      | PinNumber：[11 12 13]
      | ReadOperation：关闭
      | IOAsArray：开启
      | 是否启用仿真输入：关闭
      | 三、怎样继续学习？
      | 这是标准库子系统实例。中文说明放在使用它的父级页面，并同步存入本块Descriptio
      | n（模块说明）；官方库链接保留。先看本实例的输入来自哪里、输出交给谁，再结合
      | 以上参数理解作用。
  note: 【本页库子系统中文说明】GPIOE_三路阀反馈
      | 一、它做什么？
      | 这是官方数字端口读取块，读取指定GPIO端口/引脚当前的高低电平，再交给输入映射
      | 模块解释为反馈或告警。高电平不必然代表“正常”或“开启”，要结合电路极性和后
      | 面的取反逻辑。它只读反馈，不在这里产生输出驱动。
      | 二、本实例当前参数
      | 端口名称：GPIOE
      | PinNumber：[13 14 15]
      | ReadOperation：开启
      | IOAsArray：开启
      | 采样时间（秒）：0.001
      | 是否启用仿真输入：关闭
      | 三、怎样继续学习？
      | 这是标准库子系统实例。中文说明放在使用它的父级页面，并同步存入本块Descriptio
      | n（模块说明）；官方库链接保留。先看本实例的输入来自哪里、输出交给谁，再结合
      | 以上参数理解作用。
  note: 【本页库子系统中文说明】GPIOE_阀驱动输出
      | 一、它做什么？
      | 这是官方数字端口写入块，把模型传来的高低电平写到已配置的GPIO端口。前面的Boar
      | dOutput已处理周期、使能和电平极性，这里负责真正交给硬件；板级引脚初始化由Cub
      | eMX生成。软件值与阀门的通断关系取决于外部电路，不应仅凭0或1猜动作。
      | 二、本实例当前参数
      | 端口名称：GPIOE
      | PinNumber：[7 8 10]
      | ReadOperation：关闭
      | IOAsArray：开启
      | 是否启用仿真输入：关闭
      | 三、怎样继续学习？
      | 这是标准库子系统实例。中文说明放在使用它的父级页面，并同步存入本块Descriptio
      | n（模块说明）；官方库链接保留。先看本实例的输入来自哪里、输出交给谁，再结合
      | 以上参数理解作用。
  note: 【中文功能与算法导航】
      | 本轮覆盖259个子系统实例：189个自定义实现、70个库实例。
      | 双击普通子系统：查看右侧功能、公式和输入输出说明。
      | 打开Stateflow图：查看功能面板，迁移Description说明判据及动作。
      | 打开MATLAB函数：代码头部说明功能及关键公式。
      | 库实例说明在父页面和实例Description中，库链接保留。
      | 连线Description说明数据用途；关键温压计算线另有可见标签。
      | 完整资料：20261030/子系统功能与算法说明.md、连线功能说明.csv。
      | 阅读顺序：BoardInput → COMMRead_ISM → ESM → CLM → ControlOut → BoardOutput。
      | 辅助功能：FPM/MAM/SDM为保护告警；SaveData/SendData为记录回传；FRAM为双区保存与复位恢复。
  note: ADC1_八路采样
      | ADC1八路采样：把模拟电压变成八个原始计数
      |
      | ADC1按0.02 s（20 ms）执行一次常规组触发和读取，输出8项计数，未启用多组缓冲。数组顺序依次为
      | CH2/PA2电源、CH3/PA3预留、内部温度传感器、CH4/PA4排温、CH5/PA5总温参考、CH6/PA6预留、CH8/P
      | B0总温测量、CH9/PB1油压。
      |
      | 这些输出首先是ADC计数，不是伏特或摄氏度。BoardInput/In06把电源换成电压，转交排温/油压/芯片
      | 温度计数，并计算总温编码；ISM随后标定、滤波，才得到控制和记录采用的量。
      |
      | 例如电源计数2048经In06的2048×48/4096得到24 V；但不能把同一系数套用到排温或油压。第2、6路当
      | 前没有进入有效模拟量处理。
  note: GPIOD_PD8_Alarm
      | GPIOD_PD8_Alarm：读取GPIOD第8号引脚的数字电平
      |
      | 采样周期0.001 s，输出单个引脚的0/1原始电平。本实例只读一个引脚，避免多引脚输出维度与仿真返
      | 回标量不一致。
      |
      | PD8、PD9进入告警/状态输入整理。电平是否代表有效，要继续看BoardInput中的逻辑取反与组合，不
      | 能只凭读到1就说阀门已经打开。本处没有去抖、延时确认或模拟量换算。
  note: GPIOD_PD9_Alarm
      | GPIOD_PD9_Alarm：读取GPIOD第9号引脚的数字电平
      |
      | 采样周期0.001 s，输出单个引脚的0/1原始电平。本实例只读一个引脚，避免多引脚输出维度与仿真返
      | 回标量不一致。
      |
      | PD8、PD9进入告警/状态输入整理。电平是否代表有效，要继续看BoardInput中的逻辑取反与组合，不
      | 能只凭读到1就说阀门已经打开。本处没有去抖、延时确认或模拟量换算。
  note: GPIOD_使能镜像点火
      | GPIOD_使能镜像点火：把已计算好的电平写到硬件输出脚
      |
      | 输入数组按引脚顺序写入GPIOD [11 12 13]，是一项对应一个引脚，不能改变排列。
      |
      | PD11对应主阀使能、PD12对应主阀开通镜像、PD13对应点火输出。周期和开通时间已在BoardOutput时
      | 序层计算，本处只写电平，不重新做PWM，也不读取阀门实际动作。
      |
      | 输出电平是命令，输入侧GPIO反馈是另一条独立链路；两者数值相同不自动证明机械动作正常。
  note: GPIOE_PE13_Feedback
      | GPIOE_PE13_Feedback：读取GPIOE第13号引脚的数字电平
      |
      | 采样周期0.001 s，输出单个引脚的0/1原始电平。本实例只读一个引脚，避免多引脚输出维度与仿真返
      | 回标量不一致。
      |
      | PE13、PE14、PE15分别进入三路阀反馈整理。电平是否代表有效，要继续看BoardInput中的逻辑取反与
      | 组合，不能只凭读到1就说阀门已经打开。本处没有去抖、延时确认或模拟量换算。
  note: GPIOE_PE14_Feedback
      | GPIOE_PE14_Feedback：读取GPIOE第14号引脚的数字电平
      |
      | 采样周期0.001 s，输出单个引脚的0/1原始电平。本实例只读一个引脚，避免多引脚输出维度与仿真返
      | 回标量不一致。
      |
      | PE13、PE14、PE15分别进入三路阀反馈整理。电平是否代表有效，要继续看BoardInput中的逻辑取反与
      | 组合，不能只凭读到1就说阀门已经打开。本处没有去抖、延时确认或模拟量换算。
  note: GPIOE_PE15_Feedback
      | GPIOE_PE15_Feedback：读取GPIOE第15号引脚的数字电平
      |
      | 采样周期0.001 s，输出单个引脚的0/1原始电平。本实例只读一个引脚，避免多引脚输出维度与仿真返
      | 回标量不一致。
      |
      | PE13、PE14、PE15分别进入三路阀反馈整理。电平是否代表有效，要继续看BoardInput中的逻辑取反与
      | 组合，不能只凭读到1就说阀门已经打开。本处没有去抖、延时确认或模拟量换算。
  note: GPIOE_阀驱动输出
      | GPIOE_阀驱动输出：把已计算好的电平写到硬件输出脚
      |
      | 输入数组按引脚顺序写入GPIOE [7 8 10]，是一项对应一个引脚，不能改变排列。
      |
      | PE7对应副油阀、PE8对应主油阀、PE10对应引气阀，父级已生成相应有效电平。周期和开通时间已在Bo
      | ardOutput时序层计算，本处只写电平，不重新做PWM，也不读取阀门实际动作。
      |
      | 输出电平是命令，输入侧GPIO反馈是另一条独立链路；两者数值相同不自动证明机械动作正常。
  ADC1_八路采样 : stm32f4xxblockslib/Analog to Digital Converter  Description=|  ADCModule=ADC1  ConversionGroup=Regular  TriggerMode=Trigger and read  NumberOfConversions=8  EnableBufferConv=off  BufferLength=1  OutputStatus=off  SampleTime=0.02  EnableSimPort=off  hoistedMaskSrc=ECSoC/ECSimCodegen/Analog to Digital Converter
      | ADC1八路采样：把模拟电压变成八个原始计数
      | 
      | ADC1按0.02 s（20 ms）执行一次常规组触发和读取，输出8项计数，未启用多组缓冲。数组顺序依次为CH2/PA2电源、CH3/PA3预留、内部温度传感器、CH4/PA4排温、CH5/PA5总温参考、CH6/PA6预留、CH8/PB0总温测量、CH9/PB1油压。
      | 
      | 这些输出首先是ADC计数，不是伏特或摄氏度。BoardInput/In06把电源换成电压，转交排温/油压/芯片温度计数，并计算总温编码；ISM随后标定、滤波，才得到控制和记录采用的量。
      | 
      | 例如电源计数2048经In06的2048×48/4096得到24 V；但不能把同一系数套用到排温或油压。第2、6路当前没有进入有效模拟量处理。
  BoardInput_输入换算与协议解析 : Subsystem  Description=|  TreatAsAtomicUnit=on  SystemSampleTime=0.001
      | 板级输入怎样交给控制算法
      | 
      | 这里是硬件与控制算法之间的输入整理层，父级每1 ms调用。外面已经读到了ADC数组、三路串口字节、数字端口和定时器捕获值；本层把不同来源整理成固定输出，让下游不用直接处理零散字节和电平。
      | 
      | 上位机字节进入In01_Host，找到AA55帧头，收齐14字节并通过累加/异或校验后，保持最新命令数组，按20 ms节拍通知控制算法。
      | 电机字节进入In02_Motor，收齐9字节、CRC正确后计算电机转速。In03_Pump保留22字节油泵回包校验，但这个输入侧预留结果不参与实际泵速回传；实际泵反馈处理在BoardOutput/Out01_Pump。
      | 
      | 定时器数据先到In04_Capture，用相邻计数差建立最近10项间隔缓存；再到In05_Speed，以电机反馈和捕获估算两种来源选出控制转速。控制转速每20 ms更新，其余毫秒保持。
      | 
      | ADC数据进入In06_Analog：第1项换电源电压，第3、4、8项转交芯片温度/排温/油压计数，第5和7项一起反算总温，第2和6项暂未使用。
      | GPIOE/GPIOD进入In07_GPIO，按硬件电平极性映射成五个反馈；FRAM通知和20字节内容由In08_FRAM转交。
      | 
      | 输出再经过根层ControlRate送入COMMRead_ISM。注意本层多数温度和油压仍是原始计数，下游ISM才做标定滤波；父级1 ms调用不等于所有传感器每1 ms获得新采样。
  BoardOutput_串口封装与阀门时序 : Subsystem  Description=|  TreatAsAtomicUnit=on  SystemSampleTime=0.001
      | 控制要求怎样变成板上的电平与串口帧
      | 
      | 上层ControlOut给出油泵、电机、阀门、点火等要求，SendData给出回传协议字段。本层按1 ms任务运行，把这些要求变成外层STM32驱动块能直接接收的数据，而不是重新决定发动机处于哪种控制模式。
      | 
      | Out01_Pump接收油泵串口回包，校验22字节帧并平滑泵速，用于回传。
      | Out02_Timing把主副阀的周期与开通计数变成开关节奏，再按电路低有效极性形成GPIOE/GPIOD输出；点火请求形成9 ms开、1 ms关的循环。
      | 
      | Out03_Telemetry按20 ms节拍，将回传字段、帧号和实际泵速排成28字节内容，再追加两项校验，形成30字节上位机帧。
      | Out04_Command按20 ms节拍生成两路9字节外设帧。电机命令高字节固定0，油泵命令使用原高低给定字节，CRC只覆盖两个命令字节。
      | 
      | Out05_Handoff集中转交电平、三路串口帧和有效长度，并处理软件复位请求。实际UART/GPIO动作发生在根层官方硬件块中；生成一帧数据不等于串口已经物理发送完成。
  Bus Creator1 : BusCreator  Inputs=25  OutDataTypeStr=Bus: SaveData_Out  NonVirtualBus=on
      settings: AttributesFormatString=Bus Creator1（25项运行记录总线）  InheritFromInputs=off
  Bus Creator2 : BusCreator  Inputs=18  OutDataTypeStr=Bus: EngineControl_Out  NonVirtualBus=on
      settings: AttributesFormatString=Bus Creator2（18项执行控制总线）  InheritFromInputs=off
  Bus Creator3 : BusCreator  Inputs=29  OutDataTypeStr=Bus: SendData_Out  NonVirtualBus=on
      settings: AttributesFormatString=Bus Creator3（29字段回传及外设命令总线）  InheritFromInputs=off
  Bus Selector4 : BusSelector  OutputSignals=ServoCtrlFlag（执行控制状态标志）
      settings: AttributesFormatString=Bus Selector4（总线选择器4）
  CLM : Subsystem  Description=|  RequirementInfo={} %GIDa_551bc864_6ae2_4221_b439_5f222ab60bd4  TreatAsAtomicUnit=on  SystemSampleTime=0.02
      | 发动机当前模式怎样选出一套执行要求
      | 
      | ESM给本层EngineState，决定这次启用原位Origin、普通起动Start、闭环ClpControl、手动Manual或停车Stop中的哪一支。每支先生成自己的油泵、阀门、电机与点火候选值，不是同时把五套结果送硬件。
      | 
      | 原位分支还计算进入起动前的温度和油压参考；普通起动分支用这些初始条件推进开环时序；闭环分支根据目标与反馈转速修正油泵给定；手动分支响应上位机设置；停车分支产生停车过程要求。
      | 各分支通过Merge交接当前控制模式和进度，不应把非当前分支的保持值当成刚计算的新要求。
      | 
      | ControlOut_Manage最后统一仲裁：油泵给定按模式选择并限幅，阀门/电机/点火等字段按对应模式选择。结果组成S_Servo_Out，送ControlOut再到BoardOutput生成物理电平和串口帧。
      | 
      | 上一周期执行输出和原位参考通过延迟回到本层，供增量PI、手动保持和初始值锁存使用。当前输入与上一周期值是不同用途，删掉记忆反馈会改变算法。当前只保留普通Start，已没有AirStart/BWStart分支。
      settings: AttributesFormatString=CLM（控制规律管理）  OpenFcn=open_system(gcbh,'force');
      mask Display:
      | port_label('input',1,'S_SPM（输入综合信息）','texmode','off');
      | port_label('input',2,'S_EngineState（发动机状态）','texmode','off');
      | port_label('input',3,'S_FAM（故障标志）','texmode','off');
      | port_label('output',1,'S_Servo_Out（执行控制总线）','texmode','off');
      | port_label('output',2,'S_ClM_Parameter（控制规律参数）','texmode','off');
  COMMRead_ISM : Subsystem  Description=|  RequirementInfo={} %GIDa_b97d35a5_fe89_4d5d_88b1_95feecd683f6  Priority=0  TreatAsAtomicUnit=on  SystemSampleTime=0.02
      | 把通信输入和板载采样整理成控制器可用的数据
      | 
      | 这是输入侧的汇合处。CMMRead负责解释上位机命令、目标转速、环境和飞行信息；ISM负责把板载ADC与测速数据标定、筛选、滤波，输出传感器总线。两类来源分开保留，名称相近也不代表同一测量。
      | 
      | 例如ADC供电电压用于监视与回传，而通信中的V_Power来自上位机字段；排温经过标定、低通后进入起动及告警。温度修正转速另用于记录和回传，不应与闭环采用的Nc_Filter混用。
      | 
      | 内部还有复位记录解码接口，但当前恢复使能接常量false，外部FRAM有效标志未实际投入这条恢复选择。Dynamic_Cal虽然计算总温总压，送到ISM转速修正接口的T1t当前仍为288.15 K常量。注释按现有连接说明，不能把预留算法当作已投入功能。
      settings: AttributesFormatString=COMMRead_ISM（飞发通信解析与信号管理）  OpenFcn=open_system(gcbh,'force');
      mask Display:
      | port_label('input',1,'S_Flag_rx_suc（指令帧有效）','texmode','off');
      | port_label('input',2,'S_PF_MyUsart2_Rxdata（四号串口指令数据）','texmode','off');
      | port_label('input',3,'S_Flag_ECUReset（复位恢复标志）','texmode','off');
      | port_label('input',4,'S_ECUReset_Information（复位恢复记录）','texmode','off');
      | port_label('input',5,'S_MySet_Rxdata（配置数据）','texmode','off');
      | port_label('input',6,'S_Nc（反馈转速）','texmode','off');
      | port_label('input',7,'S_T4（排温采样码）','texmode','off');
      | port_label('input',8,'S_Vpower（电源电压）','texmode','off');
      | port_label('input',9,'S_Tecu（处理器温度码）','texmode','off');
      | port_label('input',10,'S_SWI_Firework（点火器报警反馈）','texmode','off');
      | port_label('input',11,'S_SWI_EValve（主油阀反馈）','texmode','off');
      | port_label('input',12,'S_SWI_Eblast（副油阀反馈）','texmode','off');
      | port_label('input',13,'S_SWI_ValveErr（阀报警反馈）','texmode','off');
      | port_label('input',14,'S_EngineState（发动机状态）','texmode','off');
      | port_label('input',15,'S_SWI_BleedAir（引气阀反馈）','texmode','off');
      | port_label('input',16,'S_POil（油压输入，单位待核）','texmode','off');
      | port_label('input',17,'S_T0（总温编码）','texmode','off');
      | port_label('output',1,'S_SPM（输入综合信息）','texmode','off');
  Clock_模型时钟 : DigitalClock  SampleTime=0.001
  ControlOut : Subsystem  Description=|  TreatAsAtomicUnit=on  SystemSampleTime=0.02
      | 把选定的控制结果整理为执行接口
      | 
      | 接收控制模式已经选好的油泵、阀门、电机和开关量，按输出总线规定的字段顺序整理，供BoardOutput统一执行。这里不重新计算目标转速，也不把各模式的控制结果相加。
      | 
      | 数值控制量和使能需要一起理解：阀门有周期、开通计数及使能，电机同样有自己的允许条件；油泵给定还会被转换为通信命令。输出的控制编码不是执行器反馈，实际转速和阀门反馈由独立输入链路返回。
      | 
      | 从此处继续追线到BoardOutput，才会看到2 ms时序、UART帧以及GPIO有效电平。
      settings: AttributesFormatString=ControlOut（执行控制接口）  OpenFcn=open_system(gcbh,'force');
      mask Display:
      | port_label('input',1,'S_EngineState（发动机状态）','texmode','off');
      | port_label('input',2,'S_Servo_Out（执行控制总线）','texmode','off');
      | port_label('input',3,'S_SPM（输入综合信息）','texmode','off');
      | port_label('input',4,'S_FAM（故障标志）','texmode','off');
      | port_label('output',1,'Out_EValve_Cycle（主油阀周期）','texmode','off');
      | port_label('output',2,'Out_EValve_Open（主油阀开通）','texmode','off');
      | port_label('output',3,'Out_Eblast_Cycle（副油阀周期）','texmode','off');
      | port_label('output',4,'Out_Eblast_Open（副油阀开通）','texmode','off');
      | port_label('output',5,'Out_Motor_Cycle（起动电机周期计数）','texmode','off');
      | port_label('output',6,'Out_Motor_Open（起动电机开通计数）','texmode','off');
      | port_label('output',7,'Out_EValve_Enable（主油阀使能）','texmode','off');
      | port_label('output',8,'Out_Eblast_Enable（副油阀使能）','texmode','off');
      | port_label('output',9,'Out_Motor_Enable（起动电机使能）','texmode','off');
      | port_label('output',10,'Out_SWO_Firework（点火器使能）','texmode','off');
      | port_label('output',11,'Out_SWO_BleedAir（引气阀使能）','texmode','off');
      | port_label('output',12,'Out_EngineState（发动机状态）','texmode','off');
      | port_label('output',13,'Out_Flag_ECUReset_Clear（清除复位恢复状态）','texmode','off');
      | port_label('output',14,'Out_Flag_ECUReset_Save（保存复位恢复数据）','texmode','off');
      | port_label('output',15,'Out_Flag_Reset_Enable（软件复位请求）','texmode','off');
      | port_label('output',16,'Out_Accelerator（油泵给定控制量）','texmode','off');
      | port_label('output',17,'Out_Nc_dem（控制目标转速）','texmode','off');
      | port_label('output',18,'Out_Nc（反馈转速）','texmode','off');
  ControlRate10_二十毫秒输入 : RateTransition  Integrity=off  Deterministic=off  OutPortSampleTime=0.02
  ControlRate11_二十毫秒输入 : RateTransition  Integrity=off  Deterministic=off  OutPortSampleTime=0.02
  ControlRate12_二十毫秒输入 : RateTransition  Integrity=off  Deterministic=off  OutPortSampleTime=0.02
  ControlRate13_二十毫秒输入 : RateTransition  Integrity=off  Deterministic=off  OutPortSampleTime=0.02
  ControlRate14_二十毫秒输入 : RateTransition  Integrity=off  Deterministic=off  OutPortSampleTime=0.02
  ControlRate15_二十毫秒输入 : RateTransition  Integrity=off  Deterministic=off  OutPortSampleTime=0.02
  ControlRate16_二十毫秒输入 : RateTransition  Integrity=off  Deterministic=off  OutPortSampleTime=0.02
  ControlRate1_二十毫秒输入 : RateTransition  Integrity=off  Deterministic=off  OutPortSampleTime=0.02
  ControlRate2_二十毫秒输入 : RateTransition  Integrity=off  Deterministic=off  OutPortSampleTime=0.02
  ControlRate3_二十毫秒输入 : RateTransition  Integrity=off  Deterministic=off  OutPortSampleTime=0.02
  ControlRate4_二十毫秒输入 : RateTransition  Integrity=off  Deterministic=off  OutPortSampleTime=0.02
  ControlRate5_二十毫秒输入 : RateTransition  Integrity=off  Deterministic=off  OutPortSampleTime=0.02
  ControlRate6_二十毫秒输入 : RateTransition  Integrity=off  Deterministic=off  OutPortSampleTime=0.02
  ControlRate7_二十毫秒输入 : RateTransition  Integrity=off  Deterministic=off  OutPortSampleTime=0.02
  ControlRate8_二十毫秒输入 : RateTransition  Integrity=off  Deterministic=off  OutPortSampleTime=0.02
  ControlRate9_二十毫秒输入 : RateTransition  Integrity=off  Deterministic=off  OutPortSampleTime=0.02
  ESM : Subsystem  Description=|  RequirementInfo={} %GIDa_2fc1402b_e0bf_41a7_956e_2a1bb4c0c444  TreatAsAtomicUnit=on  SystemSampleTime=0.02
      | 管理发动机运行模式，而不是直接控制驱动电平
      | 
      | Flags先根据命令、当前转速、起动阶段结果、停车完成标志及恢复条件，计算允许发生哪些模式转换。StateTranslation再按当前所在模式和这些允许条件切换状态。
      | 
      | 对外只有五种运行模式：Origin=0、Start=1、Clp=2、Manual=3、Stop=4。普通起动内部的A～F及异常阶段码不属于这五个模式编号。
      | 
      | 输出EngineState供CLM选择相应控制分支，供通信与记录解释运行状态。本层不生成泵字节或GPIO脉冲；转换进入Start仅表示开始执行起动分支，不代表已达到闭环转速。
      settings: AttributesFormatString=ESM（发动机状态管理）  OpenFcn=open_system(gcbh,'force');
      mask Display:
      | port_label('input',1,'S_CLM_Parameter（控制规律参数）','texmode','off');
      | port_label('input',2,'S_SPM（输入综合信息）','texmode','off');
      | port_label('output',1,'S_EngineState（发动机状态）','texmode','off');
  FPM : Subsystem  Description=|  RequirementInfo={} %GIDa_c0e639c6_8b38_48d3_834c_1a5c30379626  TreatAsAtomicUnit=on  SystemSampleTime=0.02
      | 将测速异常和复位请求整理成控制保护标志
      | 
      | 从传感器和通信总线取得转速、故障状态、命令及运行模式。内部区分暂时的测速异常、持续故障锁存，以及恢复、清除和定期保存条件。
      | 
      | 转速超过62000的比较参与手动超速保护；ECUReset命令经Up_Hold保持，结合模式形成复位相关请求。输出FAM总线供CLM选择保持原泵值、备份供油曲线或恢复期间给定，并送FRAM事务层保存。
      | 
      | 本模块主要生成逻辑条件，不直接写FRAM或调用硬件复位。故障标志成立后的实际控制策略，在CLM/Fault_Process和输出管理中实现。
      settings: AttributesFormatString=FPM（故障处理）  OpenFcn=open_system(gcbh,'force');
      mask Display:
      | port_label('input',1,'S_SPM（输入综合信息）','texmode','off');
      | port_label('input',2,'S_EngineState（发动机状态）','texmode','off');
      | port_label('output',1,'S_FAM（故障标志）','texmode','off');
  FRAM_ControlDelay_控制快照 : UnitDelay  SampleTime=0.02  HasFrameUpgradeWarning=on
  FRAM_DataDelay_记录快照 : UnitDelay  SampleTime=0.02  HasFrameUpgradeWarning=on
  FRAM_Read_读取恢复 : Subsystem  Description=|  TreatAsAtomicUnit=on
      | 在发送允许时完成67字节FRAM读写传输
      | 
      | 输入为Step06生成的67字节SPI帧。Enable允许时才执行SPI2传输；读帧先发送03和两字节地址，再用64个占位字节产生时钟，返回帧中的后64字节才是记录。
      | 
      | 该接口也用于整条记录写入：写帧为02、地址高、地址低和64字节数据。SPI采用模式3。返回帧经上层延迟交事务模块检查，不在本模块判断CRC或决定恢复。
      | 
      | 名称含“读取恢复”，但实际帧的操作码决定读还是写；不能只凭模块名称认定其永远只读。没有使能时不会每拍重新访问FRAM。
  FRAM_RxDelay_传输反馈 : UnitDelay  SampleTime=0.001  HasFrameUpgradeWarning=on
  FRAM_SendDelay_协议快照 : UnitDelay  SampleTime=0.02  HasFrameUpgradeWarning=on
  FRAM_使能返回终止 : Terminator
  FRAM_写使能命令 : Subsystem  Description=|  TreatAsAtomicUnit=on
      | 给FRAM发送一字节写使能命令
      | 
      | Enable有效时，通过SPI2模式3发送输入的单字节命令，正常为06。FRAM后续的写入需要先取得写许可，因此事务层会在失效、整条记录写入、提交标志写入前安排它。
      | 
      | 此模块只完成写使能传输，不包含地址和数据，也不证明下一步写入成功。返回值不等于完整记录。写后是否成功，需要后面的回读与CRC检查确认。
  FRAM_四字节提交 : Subsystem  Description=|  TreatAsAtomicUnit=on
      | 单独改写FRAM记录最后的提交字节
      | 
      | 输入固定4字节：[02，地址高字节，地址低字节，写入值]。使能成立时执行一次SPI2模式3传输。地址由事务层指定为备用记录起始地址+63。
      | 
      | 先写0表示“这条记录正在更新，不可用于恢复”；完整64字节写好后，再单独写165（A5）表示“可以检查并使用”。将提交单独放最后，可避免写一半的记录被误认为完整。
      | 
      | 本模块不决定写0还是165，不选择备用区，也不计算CRC；这些由Step05、Step06安排。
  FRAM_复位恢复事务 : Subsystem  Description=|
      | 用双存储区分步保存运行快照，供复位后读取
      | 
      | FRAM首区地址0x0200，次区0x0300，每区一条64字节记录。启动先读两区，检查格式头、CRC32和最后的提交标记，再选择有效且代号较新的记录。没有有效记录时不发恢复通知。
      | 
      | 运行中收到保存/清除请求，且空闲、间隔达到0.5 s或模式已变化时，冻结本次快照。新记录写到备用区：先把提交字节写0，再写完整记录，最后单独把提交字节写165，回读验证成功后才切换有效区。写到一半断电时，旧有效区仍可保留。
      | 
      | 六个Step分别负责检查、选择、请求、打包、推进状态和生成命令。StateMemory保存上一拍事务状态；本拍发出的SPI命令，其返回帧要到后续拍再使用，不是在一段函数里同步完成全部读写。
      | 
      | 恢复内容20字节包括泵给定、发动机状态、目标/实际转速等关键字段，不是保存所有ADC通道。Errors只累计写后验证失败。恢复通知对齐20 ms边界且每次启动只发一次；下游当前恢复使用使能未接通，不能把“此处有恢复通知”当成整机已恢复执行。
  FRAM_提交返回终止 : Terminator
  GPIOD_AlarmVector : Mux  Inputs=2
  GPIOD_PD8_Alarm : stm32f4xxblockslib/Digital Port Read  Description=|  PortName=GPIOD  PinNumber=8  ReadOperation=on  IOAsArray=on  SampleTime=0.001  EnableSimPort=off  hoistedMaskSrc=ECSoC/ECSimCodegen/Digital Port Read
      | GPIOD_PD8_Alarm：读取GPIOD第8号引脚的数字电平
      | 
      | 采样周期0.001 s，输出单个引脚的0/1原始电平。本实例只读一个引脚，避免多引脚输出维度与仿真返回标量不一致。
      | 
      | PD8、PD9进入告警/状态输入整理。电平是否代表有效，要继续看BoardInput中的逻辑取反与组合，不能只凭读到1就说阀门已经打开。本处没有去抖、延时确认或模拟量换算。
  GPIOD_PD9_Alarm : stm32f4xxblockslib/Digital Port Read  Description=|  PortName=GPIOD  PinNumber=9  ReadOperation=on  IOAsArray=on  SampleTime=0.001  EnableSimPort=off  hoistedMaskSrc=ECSoC/ECSimCodegen/Digital Port Read
      | GPIOD_PD9_Alarm：读取GPIOD第9号引脚的数字电平
      | 
      | 采样周期0.001 s，输出单个引脚的0/1原始电平。本实例只读一个引脚，避免多引脚输出维度与仿真返回标量不一致。
      | 
      | PD8、PD9进入告警/状态输入整理。电平是否代表有效，要继续看BoardInput中的逻辑取反与组合，不能只凭读到1就说阀门已经打开。本处没有去抖、延时确认或模拟量换算。
  GPIOD_使能镜像点火 : stm32f4xxblockslib/Digital Port Write  Description=|  PortName=GPIOD  PinNumber=[11 12 13]  ReadOperation=off  IOAsArray=on  EnableSimPort=off  hoistedMaskSrc=ECSoC/ECSimCodegen/Digital Port Write
      | GPIOD_使能镜像点火：把已计算好的电平写到硬件输出脚
      | 
      | 输入数组按引脚顺序写入GPIOD [11 12 13]，是一项对应一个引脚，不能改变排列。
      | 
      | PD11对应主阀使能、PD12对应主阀开通镜像、PD13对应点火输出。周期和开通时间已在BoardOutput时序层计算，本处只写电平，不重新做PWM，也不读取阀门实际动作。
      | 
      | 输出电平是命令，输入侧GPIO反馈是另一条独立链路；两者数值相同不自动证明机械动作正常。
  GPIOE_FeedbackVector : Mux  Inputs=3
  GPIOE_PE13_Feedback : stm32f4xxblockslib/Digital Port Read  Description=|  PortName=GPIOE  PinNumber=13  ReadOperation=on  IOAsArray=on  SampleTime=0.001  EnableSimPort=off  hoistedMaskSrc=ECSoC/ECSimCodegen/Digital Port Read
      | GPIOE_PE13_Feedback：读取GPIOE第13号引脚的数字电平
      | 
      | 采样周期0.001 s，输出单个引脚的0/1原始电平。本实例只读一个引脚，避免多引脚输出维度与仿真返回标量不一致。
      | 
      | PE13、PE14、PE15分别进入三路阀反馈整理。电平是否代表有效，要继续看BoardInput中的逻辑取反与组合，不能只凭读到1就说阀门已经打开。本处没有去抖、延时确认或模拟量换算。
  GPIOE_PE14_Feedback : stm32f4xxblockslib/Digital Port Read  Description=|  PortName=GPIOE  PinNumber=14  ReadOperation=on  IOAsArray=on  SampleTime=0.001  EnableSimPort=off  hoistedMaskSrc=ECSoC/ECSimCodegen/Digital Port Read
      | GPIOE_PE14_Feedback：读取GPIOE第14号引脚的数字电平
      | 
      | 采样周期0.001 s，输出单个引脚的0/1原始电平。本实例只读一个引脚，避免多引脚输出维度与仿真返回标量不一致。
      | 
      | PE13、PE14、PE15分别进入三路阀反馈整理。电平是否代表有效，要继续看BoardInput中的逻辑取反与组合，不能只凭读到1就说阀门已经打开。本处没有去抖、延时确认或模拟量换算。
  GPIOE_PE15_Feedback : stm32f4xxblockslib/Digital Port Read  Description=|  PortName=GPIOE  PinNumber=15  ReadOperation=on  IOAsArray=on  SampleTime=0.001  EnableSimPort=off  hoistedMaskSrc=ECSoC/ECSimCodegen/Digital Port Read
      | GPIOE_PE15_Feedback：读取GPIOE第15号引脚的数字电平
      | 
      | 采样周期0.001 s，输出单个引脚的0/1原始电平。本实例只读一个引脚，避免多引脚输出维度与仿真返回标量不一致。
      | 
      | PE13、PE14、PE15分别进入三路阀反馈整理。电平是否代表有效，要继续看BoardInput中的逻辑取反与组合，不能只凭读到1就说阀门已经打开。本处没有去抖、延时确认或模拟量换算。
  GPIOE_阀驱动输出 : stm32f4xxblockslib/Digital Port Write  Description=|  PortName=GPIOE  PinNumber=[7 8 10]  ReadOperation=off  IOAsArray=on  EnableSimPort=off  hoistedMaskSrc=ECSoC/ECSimCodegen/Digital Port Write
      | GPIOE_阀驱动输出：把已计算好的电平写到硬件输出脚
      | 
      | 输入数组按引脚顺序写入GPIOE [7 8 10]，是一项对应一个引脚，不能改变排列。
      | 
      | PE7对应副油阀、PE8对应主油阀、PE10对应引气阀，父级已生成相应有效电平。周期和开通时间已在BoardOutput时序层计算，本处只写电平，不重新做PWM，也不读取阀门实际动作。
      | 
      | 输出电平是命令，输入侧GPIO反馈是另一条独立链路；两者数值相同不自动证明机械动作正常。
  LogErrors_恢复错误记录 : RateTransition  Integrity=off  Deterministic=off  OutPortSampleTime=0.02
  LogPack_运行记录列定义 : Subsystem  Description=|
      | 给运行日志规定固定的27列顺序
      | 
      | 把SaveData的25项数据、当前秒数及FRAM写后验证失败次数合并为27×1的single列向量。固定列序让不同采样时刻可以按同一含义解释，不应把它当作27字节通信帧。
      | 
      | 这些值仍按各自记录编码保存，并非全部是国际单位制物理量。温度、压力、转速、模式和版本字段的意义不同，部分项在SaveData中已经做过比例缩放。
      | 
      | 输出到SDLog的To Workspace，仿真得到engine_log。名称中的日志/SD不表示本模块已经把数据可靠落到实际SD卡；实际存储行为由外部记录接口决定。
  LogTime_记录时钟 : RateTransition  Integrity=off  Deterministic=off  OutPortSampleTime=0.02
  MAM : Subsystem  Description=|  TreatAsAtomicUnit=on  SystemSampleTime=0.02
      | 生成排温、转速和供电相关的监视告警
      | 
      | 读取传感器总线。滤波排温T4_Filter超过850后需要定时确认；转速超过62000 rpm也需要定时确认，两条确认时间均约2 s。这样短暂一拍越限不会立即作为持续超限输出。
      | 
      | ADC换算的供电电压低于22 V参与欠压判断，这条支路没有相同的2 s持续确认。告警结果打成监视总线，供状态回传等下游使用。
      | 
      | 告警标志不等于本模块已经执行停车。是否切换运行模式或修改驱动，要继续查看相关标志的实际去向；本模块自身没有直接发送油泵零命令或关闭GPIO。
      settings: AttributesFormatString=MAM（监控报警）  OpenFcn=open_system(gcbh,'force');
      mask Display:
      | port_label('input',1,'S_ServoCtrlFlag（油泵给定选择）','texmode','off');
      | port_label('input',2,'S_FPM（故障处理信息）','texmode','off');
      | port_label('input',3,'S_SPM（输入综合信息）','texmode','off');
      | port_label('input',4,'EngineState（发动机状态）','texmode','off');
      | port_label('output',1,'S_MAlarm（监控告警）','texmode','off');
  PreviousControl_上一周期控制 : UnitDelay  SampleTime=0.02  HasFrameUpgradeWarning=on
  SDLog_官方SD卡记录 : ToWorkspace  VariableName=engine_log  SampleTime=0.02
      settings: MaxDataPoints=128
  SDM : Subsystem  Description=|  RequirementInfo={} %GIDa_6d95827b_cded_4a00_8179_e811e0d0ac4a  TreatAsAtomicUnit=on  SystemSampleTime=0.02
      | 根据运行阶段组合检测标志；当前结果未参与模式控制
      | 
      | 内部包含排温检查和逻辑选择，依据初始模式、起动相关条件组合出检测结果。T4_Check比较排温是否超过100，帮助区分尚冷与已经升温的状态。
      | 
      | 需要注意实际去向：S_SDM送到SendData后接Unused_SDM终止端，当前没有由这条输出进一步驱动ESM起动/停车转换。这里算出了检测量，不代表它已经参与发动机状态控制。
      | 
      | 实际模式转换由ESM/Flags及StateTranslation决定。阅读本模块时应将“检测算法存在”和“检测结果被控制器使用”分开。
      settings: AttributesFormatString=SDM（传感器自检与状态数据）  OpenFcn=open_system(gcbh,'force');
      mask Display:
      | port_label('input',1,'S_SPM（输入综合信息）','texmode','off');
      | port_label('input',2,'S_EngineState（发动机状态）','texmode','off');
      | port_label('output',1,'S_SDM（自检状态）','texmode','off');
  SaveData : Subsystem  Description=|  TreatAsAtomicUnit=on  SystemSampleTime=0.02
      | SaveData的职责：整理25项运行记录，不直接写文件
      | 
      | 从发动机模式、传感器/通信、执行输出和监视告警中取出需要记录的量，按固定25个输出端口排列，供后面的Savedata总线和LogPack使用。
      | 
      | 多数通道只转换为single，不额外加偏置、不拆高低字节。阀门和电机另计算开通比例；开关和告警另组合为位字段；Hold另产生循环序号。
      | 
      | S_ClM_Parameter输入当前直接接Terminator，未参与这些记录。第20～25项目前全部是固定0，不应沿用旧名称推断这些项已经存了主阀输出、软件版本或其他传感器量。
      | 
      | 本页没有文件路径、SD卡写入、SPI写入或串口封帧动作。它提供一组记录字段；实际数据去向还要继续看LogPack、SDLog和FRAM事务。
      | 
      | 温度、电压、油压和转速：保留数值，不按回传字节编码
      | 
      | 第2项T0取Sensor.T0，直接转single，25 ℃仍记录25，不加80。
      | 第3项dianyuandianya取Sensor.Vpower，24 V仍记录24，不乘5。
      | 第4项T4取Sensor.T4_Filter，第5项POil取Sensor.POil_Filter，保留滤波后的值，不拆成两个字节；油压单位沿用上游标定。
      | 第8项HuanSuanZhuanSu取温度修正转速，第10项WuLiZhuanSu取Sensor.Origin_Nc，保留完整转速，不除2。
      | 第16项Tecu取Sensor.Tecu，25 ℃仍记录25，不加50。
      | 第11项NBump_MuBiao取执行输出Accelerator，是泵控制给定编码，不是实测泵速。
      | 
      | 这些转换的输出类型是single。即使参数页上写有Floor，也不能据此说这里全部取整；浮点转single不等于转整数，原有小数一般仍保留到single精度。
      | 
      | 阀门和电机记录的是开通比例，不是机械反馈
      | 
      | 从S_Servo_Out取Open及Cycle，计算：
      | 第6项副油阀=100×Eblast_Open/Eblast_Cycle；
      | 第7项主油阀=100×EValve_Open/EValve_Cycle；
      | 第12项电机=100×Motor_Open/Motor_Cycle。
      | 结果转single记录，此处没有再转成uint8或强制向下取整。
      | 
      | 例周期30、开通15，记录50，代表50%开通比例；周期30、开通10，约为33.3333。它不是开了15 ms，也不是阀芯走到50%的位置。
      | 
      | 这些量来自驱动设定，使能状态另在第9项位字段里。比例非0不自动证明执行器已经动作。本页沿用原除法，没有在这里增加分母为0时的保护逻辑；本次仅更新说明。
      | 
      | 第9项开关量：命令和取反反馈合成一个数
      | 
      | 低四位来自执行输出，高四位来自传感器反馈的逻辑取反：
      | 位0，权重1：SWO_Firework点火使能；
      | 位1，权重2：EValve_Enable主阀使能；
      | 位2，权重4：Eblast_Enable副阀使能；
      | 位3，权重8：SWO_BleedAir引气使能；
      | 位4，权重16：NOT SWI_Firework；
      | 位5，权重32：NOT SWI_EValve；
      | 位6，权重64：NOT SWI_Eblast；
      | 位7，权重128：NOT SWI_BleedAir。
      | 
      | 按各位权重相加后转single存储。例只有主阀使能和取反后的主阀反馈为真，记录2+32=34。分析日志时先转成整数再按位拆解，不要把34当成开度34%。
      | 
      | Motor_Enable没有放入这8位；电机开通比例在第12项。高四位与原反馈相反，不能直接当作GPIO原电平解释。
      | 
      | 第14项告警字段：与SendData的定义存在差别
      | 
      | 各布尔量乘位权后相加，结果转single：
      | 位0（1）：Alarm_OverTemp；
      | 位1（2）：Alarm_OverSpeed；
      | 位2（4）：Flag_NcFailure；
      | 位3（8）：Alarm_ECUReset；
      | 位4（16）：Alarm_Vpower_Low；
      | 位5（32）：Sensor.SWI_ValveErr原值；
      | 位6（64）：当前常量0；
      | 位7（128）：当前常量0。
      | 
      | 例如超温、欠压为真，其余为假，得到17。这里的位5直接使用SWI_ValveErr，没有NOT；SendData对应位使用了NOT，不能拿同一套解码说明混用。这里的位6也没有接Lock_NcFailure，记录0不表示该锁存故障一定不存在。
      | 
      | 本页只组合并记录标志，不触发报警、停车或复位。判断运行状态要另外看第13项模式编号。
      | 
      | 25项顺序表：第1～13项
      | 
      | 1 ZhiLingHuiChuan：COMM.Instr_XianShi，指令回显。
      | 2 T0：入口温度，直接single。
      | 3 dianyuandianya：Sensor.Vpower，供电电压原值。
      | 4 T4：滤波后排温。
      | 5 POil：滤波后油压。
      | 6 Eblast：副油阀开通比例，100×Open/Cycle。
      | 7 EValve：主油阀开通比例，100×Open/Cycle。
      | 8 HuanSuanZhuanSu：温度修正转速完整值。
      | 9 KaiGuanLiang：命令与取反反馈的8位组合。
      | 10 WuLiZhuanSu：Sensor.Origin_Nc完整值。
      | 11 NBump_MuBiao：Accelerator泵给定控制编码。
      | 12 Motor：电机开通比例，100×Open/Cycle。
      | 13 FaDongJiZhuangTai：EngineState，0初始、1普通起动、2闭环、3手动、4停车。
      | 
      | 这些是记录项/输出端口编号，不是串口帧字节位置。第13项是发动机模式，不是指令编号或起动A～F阶段。
      | 
      | 25项顺序表：第14～25项及旧名称说明
      | 
      | 14 GuZhangXingXi：告警位组合，按本页专用位定义解码。
      | 15 zhenjishu：Hold产生的0～255循环序号。
      | 16 Tecu：Sensor.Tecu处理器温度原值，不加50。
      | 17 DianYuan：实际为COMM.SpeedLoad目标/装订转速，不是电源电压。
      | 18 H：COMM.H_Gprs导航高度，沿用输入单位，本页不作单位换算。
      | 19 speed：COMM.AirSpeed飞行空速；不是发动机轴转速。
      | 20 ZhuFaShuChu：当前固定0，不是有效主阀反馈。
      | 21 名称为12：当前固定0，此名字不表示第12项。
      | 22 BeiYong1：固定0。
      | 23 BeiYong2：固定0。
      | 24 BeiYong3：固定0。
      | 25 BeiYong4：固定0。
      | 
      | 第17项还会以savedata17被FRAM打包步骤读取，作为恢复记录中的目标转速。若把它误认为电压，会连带误读恢复信息。真正供电在第3项。
      | 
      | Hold序号与最终27项日志的关系
      | 
      | Hold每次执行时判断Out是否达到255：达到则置0，否则加1。序列循环为…253、254、255、0、1…；第15项把这个序号转single记录。
      | 
      | 它是本图执行次数的循环标记，不是时间戳。重复的序号不一定表示重复数据，因为每256次执行就回到同一编号；不要把序号差直接解释成秒数。
      | 
      | 外层LogPack按savedata1～savedata25拼接本页25项，末尾追加第26项时间（秒）和第27项FRAM写后验证失败次数，形成27×1的single向量。随后SDLog的To Workspace在仿真中生成engine_log。
      | 
      | 这里的27项是数值记录，不是27字节帧；名为SDLog也不能单凭名称断言已写入实际SD卡。实际记录周期取决于外层执行与记录接口，本页没有独立的周期触发器。
      | 
      | 读日志时不要套用SendData的还原规则
      | 
      | SaveData与SendData虽然记录同类变量，表示方式不同：
      | 日志T0直接是温度；回传T0加80。
      | 日志Tecu直接是温度；回传Tecu加50且限幅。
      | 日志电压直接是V；回传电压乘5。
      | 日志转速保留完整值；回传部分转速除2并拆字节。
      | 日志主副阀、电机比例是single，可有小数；回传比例转uint8。
      | 日志告警位5是SWI_ValveErr原值，位6为0；回传位5取反，位6接Lock_NcFailure。
      | 
      | 例如日志中T0=25、电压=24、转速=50000，应按这些数直接阅读，不能再减80、除5或乘2。开关与告警则需要按位解析，泵给定仍是控制编码。所有项统一转single不意味着所有项拥有相同单位。
      settings: AttributesFormatString=SaveData（25项运行记录输出）  OpenFcn=open_system(gcbh,'force');
      mask Display:
      | port_label('input',1,'S_EngineState（发动机状态）','texmode','off');
      | port_label('input',2,'S_SPM（输入综合信息）','texmode','off');
      | port_label('input',3,'S_ClM_Parameter（控制规律参数）','texmode','off');
      | port_label('input',4,'S_Servo_Out（执行控制总线）','texmode','off');
      | port_label('input',5,'S_MAlarm（监控告警）','texmode','off');
      | port_label('output',1,'ZhiLingHuiChuan（指令回显记录）','texmode','off');
      | port_label('output',2,'T0（总温编码）','texmode','off');
      | port_label('output',3,'dianyuandianya（电源电压记录）','texmode','off');
      | port_label('output',4,'T4（排温采样码）','texmode','off');
      | port_label('output',5,'POil（油压输入，单位待核）','texmode','off');
      | port_label('output',6,'Eblast（副油阀占空比记录）','texmode','off');
      | port_label('output',7,'EValve（主油阀占空比记录）','texmode','off');
      | port_label('output',8,'HuanSuanZhuanSu（温度修正转速记录）','texmode','off');
      | port_label('output',9,'KaiGuanLiang（开关输出及反馈位域）','texmode','off');
      | port_label('output',10,'WuLiZhuanSu（物理转速记录）','texmode','off');
      | port_label('output',11,'NBump_MuBiao（油泵目标给定原始值）','texmode','off');
      | port_label('output',12,'Motor（起动电机占空比记录）','texmode','off');
      | port_label('output',13,'FaDongJiZhuangTai（发动机状态码记录）','texmode','off');
      | port_label('output',14,'GuZhangXingXi（故障告警位域记录）','texmode','off');
      | port_label('output',15,'zhenjishu（模型记录帧序号）','texmode','off');
      | port_label('output',16,'Tecu（处理器温度码）','texmode','off');
      | port_label('output',17,'DianYuan（装订转速记录）','texmode','off');
      | port_label('output',18,'H（导航高度记录）','texmode','off');
      | port_label('output',19,'speed（飞行空速记录）','texmode','off');
      | port_label('output',20,'ZhuFaShuChu（主阀旧记录位）','texmode','off');
      | port_label('output',21,'12（第21项保留记录）','texmode','off');
      | port_label('output',22,'BeiYong1（保留记录项22）','texmode','off');
      | port_label('output',23,'BeiYong2（保留记录项23）','texmode','off');
      | port_label('output',24,'BeiYong3（保留记录项24）','texmode','off');
      | port_label('output',25,'BeiYong4（保留记录项25）','texmode','off');
  SendData : Subsystem  Description=|  TreatAsAtomicUnit=on  SystemSampleTime=0.02
      | SendData做什么：把运行量编码成回传字段
      | 
      | 本页接收传感器/通信总线、执行控制总线、发动机模式和监视告警，把它们变成回传所需的字节编码。它不直接发送UART，也不在这里生成20 ms发送节拍。
      | 
      | 29个输出端口不等于29字节串口帧：端口1是回传使能；端口2是旧协议长度常数25；端口3～27为本页提供的25个内容字段。后级Payload用AA、55、01作帧头，将端口3～27映射到帧第4～28字节，并覆盖第23、27、28字节；再追加两项校验，才形成30字节发送帧。
      | 
      | 端口28、29虽然叫NBumpH/L，在本页实际由COMM.SpeedLoad拆字节，不能称作实测泵速。真实泵速来自Out01_Pump，在后级直接覆盖帧第27、28字节。
      | 
      | S_SDM当前接Unused_SDM终止端，不参与这些内容。端口名字中的H/L表示高/低字节，编码值必须按下文比例还原，不能全部直接当作物理量。
      | 
      | 温度、供电和油压怎样编码
      | 
      | T0取Sensor.T0，先加80再向下取整转uint8：编码=floor(T0+80)。例25 ℃回传105，上位机减80还原。这里不是ADC原始计数，温度标定已在ISM完成。
      | 
      | 处理器温度取Sensor.Tecu：先加50，再限制0～255，最后向下取整转uint8。例25 ℃得到75；超出范围会截住，上位机减50只能得到截断后的温度。
      | 
      | 供电取Sensor.Vpower：编码=floor(5×电压)，例24 V得到120，解码时除5。这是ADC换算电压，不是COMM.V_Power字段。
      | 
      | T4取Sensor.T4_Filter，POil取Sensor.POil_Filter：各先向下取整转uint16，再拆成高低字节，没有在本页额外乘10。例排温500对应高1、低244；接收端按高×256+低还原500。油压单位沿用传感器标定，不能仅凭POil名称写成kPa。
      | 
      | 三类转速与泵给定，不能混作一项
      | 
      | 物理转速取Sensor.Origin_Nc，先除2；高字节=floor((转速/2)/256)，低字节=floor(转速/2) AND 255。
      | 
      | 温度修正转速取Sensor.HuanSuanZhuanSu，先除2并向下取整为uint16，再拆高低字节。它是修正后的量，不是原始脉冲计数。
      | 
      | 目标转速取COMM.SpeedLoad，也先除2，再取高低字节。例目标50000 rpm，编码25000，高97、低168；上位机合成后乘2还原50000。三条转速通道的编码步长均为2 rpm，奇数或小数部分会损失。
      | 
      | NBump_MuBiaoH/L实际取执行总线Accelerator，直接转uint16并拆字节，不除2。例泵给定3000对应高11、低184。它是控制编码，不是泵转速实测值。
      | 
      | 本页NBumpH/L取COMM.SpeedLoad直接转uint16拆分：50000会得到高195、低80。此旧接口不用于代表当前实测泵速；最终帧泵速位置由Telemetry覆盖。
      | 
      | 主阀、副阀和电机：回传开通比例
      | 
      | 读取执行控制总线中的Open和Cycle，分别计算：
      | 主油阀编码=floor(100×EValve_Open/EValve_Cycle)；
      | 副油阀编码=floor(100×Eblast_Open/Eblast_Cycle)；
      | 电机编码=floor(100×Motor_Open/Motor_Cycle)。
      | 
      | 例阀门周期30、开通15，得到50，表示50%的开通比例；不是开阀15 ms，也不是50%的机械位置。电机周期100、开通40得到40。
      | 
      | 这些量来自驱动设定，不是阀门位置传感器或实测转速。是否使能还要看开关量字段；不能只看比例非0就断言硬件正在工作。
      | 
      | 本页按原计算直接相除，没有额外在此分支添加分母保护。上游应给出正常周期值；本次只更新说明，不调整算法。
      | 
      | 开关量字节：低四位命令，高四位反馈取反
      | 
      | KaiGuanLiang把8个布尔量乘1、2、4、8、16、32、64、128后相加。位0是最低位。
      | 
      | 位0（1）：SWO_Firework点火使能；
      | 位1（2）：EValve_Enable主阀使能；
      | 位2（4）：Eblast_Enable副阀使能；
      | 位3（8）：SWO_BleedAir引气使能；
      | 位4（16）：NOT SWI_Firework；
      | 位5（32）：NOT SWI_EValve；
      | 位6（64）：NOT SWI_Eblast；
      | 位7（128）：NOT SWI_BleedAir。
      | 
      | 低四位取执行命令，高四位取传感器反馈的逻辑反值。不能把两组都解释成命令，也不能跳过NOT直接按原GPIO电平解释。
      | 
      | 例只有主阀使能和取反后的主阀反馈为真，字节为2+32=34。解码某位可用bitand(字节,该位权重)是否非0。这里未打包Motor_Enable，电机比例另走Motor端口。
      | 
      | 告警字节与发动机模式
      | 
      | GuZhangXingXi同样按位权相加：
      | 位0（1）：Alarm_OverTemp；
      | 位1（2）：Alarm_OverSpeed；
      | 位2（4）：Flag_NcFailure；
      | 位3（8）：Alarm_ECUReset；
      | 位4（16）：Alarm_Vpower_Low；
      | 位5（32）：NOT Sensor.SWI_ValveErr；
      | 位6（64）：Lock_NcFailure；
      | 位7（128）：当前常量0。
      | 
      | 例如超温和欠压同时为真，其他位为假，得到1+16=17。位5明确使用反馈取反，不能只写“阀门故障”却省略它与原反馈的反向关系。
      | 
      | FaDongJiZhuangTai直接将EngineState转uint8：0初始、1普通起动、2闭环、3手动、4停车。它不是上位机指令编号，也不是起动图A～F阶段。此处只编码，不触发告警或模式转换。
      | 
      | 输出端口1～15分别是什么
      | 
      | 1 ChuanShuBiaoZhi：固定1，供后级判断回传允许。
      | 2 ShuJuChangDu：旧协议常数25；不是最终UART发送长度。
      | 3 ZhiLingHuiChuan：COMM.Instr_XianShi转uint8。
      | 4 T0：入口温度加80的单字节编码。
      | 5 dianyuandianya：电压乘5的单字节编码。
      | 6/7 T4_H/L：排温整数高/低字节。
      | 8/9 POil_H/L：油压标定整数高/低字节。
      | 10 Eblast：副油阀开通比例百分数。
      | 11 EValve：主油阀开通比例百分数。
      | 12/13 HuanSuanZhuanSuH/L：修正转速除2后拆字节。
      | 14 KaiGuanLiang：执行开关与取反反馈的位组合。
      | 15 WuLiZhuanSuH1：物理转速除2后的高字节。
      | 
      | 本页编号是Outport序号。后级串口帧前面还有AA、55、01，因此端口3进入帧第4字节，而不是帧第3字节。
      | 
      | 输出端口16～29及后级覆盖关系
      | 
      | 16 WuLiZhuanSuL1：物理转速除2后的低字节。
      | 17/18 NBump_MuBiaoH/L：Accelerator泵给定高/低字节。
      | 19 Motor：电机开通比例百分数。
      | 20 FaDongJiZhuangTai：发动机运行模式编号。
      | 21 GuZhangXingXi：告警位组合。
      | 22 rt：本页固定0占位；后级帧第23字节改为循环帧号。
      | 23 TECU：处理器温度加50、限幅后的编码。
      | 24/25 MuBiaoZhuanSuH2/L2：目标转速除2后拆字节。
      | 26 QW、27 ER：本页固定0保留值；最终帧对应位置被真实泵速高、低字节覆盖。
      | 28/29 NBumpH/L：本页由SpeedLoad直接拆出的旧接口，不是实测泵速；Payload映射只取senddata1及3～27。
      | 
      | 最终泵反馈填入帧第27/28字节，来源为Out01_Pump滤波结果；帧第23字节由FrameCounter覆盖；最后第29/30字节是累加与异或校验。SendData自身不生成这些最终覆盖值和校验。
      | 
      | 读图时注意：编码精度与拆字节
      | 
      | 高低字节合成：整数=高字节×256+低字节。
      | 拆分16位整数：高=floor(整数/256)，低=整数 AND 255。例1000拆为3和232，不能按十进制把它拆成10和00。
      | 
      | 本页多数转换采用Floor，即向下取整。uint8仅容纳0～255，uint16容纳0～65535；除TECU已有限幅和饱和处理外，不能把每处类型转换都理解为会自动截到上下限。正常工作范围外可能发生回绕，本次未修改这些设置。
      | 
      | 比例、偏置和两字节编码都是协议表示方式，不是新的传感器标定。回传目标、执行命令、测量反馈的含义不同；判断最终线上数据还要继续看BoardOutput/Out03_Telemetry的覆盖和校验。
      settings: AttributesFormatString=SendData（29字段回传及外设命令接口）  OpenFcn=open_system(gcbh,'force');
      mask Display:
      | port_label('input',1,'S_SPM（输入综合信息）','texmode','off');
      | port_label('input',2,'S_SDM（自检状态）','texmode','off');
      | port_label('input',3,'S_Servo_Out（执行控制总线）','texmode','off');
      | port_label('input',4,'S_EngineState（发动机状态）','texmode','off');
      | port_label('input',5,'S_MAlarm（监控告警）','texmode','off');
      | port_label('output',1,'ChuanShuBiaoZhi（回传发送允许标志）','texmode','off');
      | port_label('output',2,'ShuJuChangDu（回传载荷长度25字节）','texmode','off');
      | port_label('output',3,'ZhiLingHuiChuan（回传指令回显字节）','texmode','off');
      | port_label('output',4,'T0（总温编码）','texmode','off');
      | port_label('output',5,'dianyuandianya（电源电压编码字节）','texmode','off');
      | port_label('output',6,'T4_H（排温编码高字节）','texmode','off');
      | port_label('output',7,'T4_L（排温编码低字节）','texmode','off');
      | port_label('output',8,'POil_H（燃油压力编码高字节）','texmode','off');
      | port_label('output',9,'POil_L（燃油压力编码低字节）','texmode','off');
      | port_label('output',10,'Eblast（副油阀占空比字节）','texmode','off');
      | port_label('output',11,'EValve（主油阀占空比字节）','texmode','off');
      | port_label('output',12,'HuanSuanZhuanSuH（修正转速编码高字节）','texmode','off');
      | port_label('output',13,'HuanSuanZhuanSuL（修正转速编码低字节）','texmode','off');
      | port_label('output',14,'KaiGuanLiang（驱动及反馈状态位域）','texmode','off');
      | port_label('output',15,'WuLiZhuanSuH1（物理转速编码高字节）','texmode','off');
      | port_label('output',16,'WuLiZhuanSuL1（物理转速编码低字节）','texmode','off');
      | port_label('output',17,'NBump_MuBiaoH（油泵目标给定高字节）','texmode','off');
      | port_label('output',18,'NBump_MuBiaoL（油泵目标给定低字节）','texmode','off');
      | port_label('output',19,'Motor（起动电机占空比命令）','texmode','off');
      | port_label('output',20,'FaDongJiZhuangTai（发动机状态码字节）','texmode','off');
      | port_label('output',21,'GuZhangXingXi（故障告警位域字节）','texmode','off');
      | port_label('output',22,'rt（帧序号占位）','texmode','off');
      | port_label('output',23,'TECU（处理器温度编码）','texmode','off');
      | port_label('output',24,'MuBiaoiZhuanSuH2（控制目标转速编码高字节）','texmode','off');
      | port_label('output',25,'MuBiaoZhuanSuL2（控制目标转速编码低字节）','texmode','off');
      | port_label('output',26,'QW（占位字节）','texmode','off');
      | port_label('output',27,'ER（占位字节）','texmode','off');
      | port_label('output',28,'NBumpH（装订转速高字节）','texmode','off');
      | port_label('output',29,'NBumpL（装订转速低字节）','texmode','off');
  TIM3_转速边沿捕获 : stm32blockslib/Timer Capture  TimerModule=TIM3  SelectedChannel=CH2  CaptureLength=16  OutputDataLength=on  OutputOverrunStatus=off  OutputDirection=off  SampleTime=0.001
      settings: LibrarySourceBlock=stm32f4xxblockslib/Timer Capture
  Time Delay2 : UnitDelay  SampleTime=-1  HasFrameUpgradeWarning=on
      settings: AttributesFormatString=Time Delay2（时间延迟2）
  UART4_发送协议帧 : stm32blockslib/UART//USART Write  UARTModule=UART4  LengthOfDataToSend=on  BlockingMode=off  BlockingTimeout=0.1  OutputStatus=off
      settings: LibrarySourceBlock=stm32f4xxblockslib/UART//USART Write
  UART4_接收字节流 : stm32blockslib/UART//USART Read  UARTModule=UART4  DataType=uint8  DataLength=64  BlockingMode=off  BlockingTimeout=0.1  OutputLength=on  OutputStatus=off  SampleTime=0.001
      settings: LibrarySourceBlock=stm32f4xxblockslib/UART//USART Read
  USART1_发送协议帧 : stm32blockslib/UART//USART Write  UARTModule=USART1  LengthOfDataToSend=on  BlockingMode=off  BlockingTimeout=0.1  OutputStatus=off
      settings: LibrarySourceBlock=stm32f4xxblockslib/UART//USART Write
  USART1_接收字节流 : stm32blockslib/UART//USART Read  UARTModule=USART1  DataType=uint8  DataLength=64  BlockingMode=off  BlockingTimeout=0.1  OutputLength=on  OutputStatus=off  SampleTime=0.001
      settings: LibrarySourceBlock=stm32f4xxblockslib/UART//USART Read
  USART2_发送协议帧 : stm32blockslib/UART//USART Write  UARTModule=USART2  LengthOfDataToSend=on  BlockingMode=off  BlockingTimeout=0.1  OutputStatus=off
      settings: LibrarySourceBlock=stm32f4xxblockslib/UART//USART Write
  USART2_接收字节流 : stm32blockslib/UART//USART Read  UARTModule=USART2  DataType=uint8  DataLength=64  BlockingMode=off  BlockingTimeout=0.1  OutputLength=on  OutputStatus=off  SampleTime=0.001
      settings: LibrarySourceBlock=stm32f4xxblockslib/UART//USART Read
  Controldata : Outport
      settings: AttributesFormatString=Controldata（18项执行控制输出）
  savedata : Outport  Port=2
      settings: AttributesFormatString=savedata（25项运行记录输出）
  senddata : Outport  Port=3
      settings: AttributesFormatString=senddata（29字段回传及外设命令接口）
  wires:
  ESM/1(S_EngineState) -> [EngineState]  "EngineState（发动机状态）"
  FPM/1(S_FAM) -> [FAM], MAM/2(S_FPM), CLM/3(S_FAM)  "FAM（故障标志）"
  [EngineState] -> CLM/2(S_EngineState)
  MAM/1(S_MAlarm) -> [MAlarm]  "MAlarm（监控告警）"
  CLM/1(S_Servo_Out) -> [S_Servo_Out]  "S_Servo_Out（执行控制总线）"
  SDM/1(S_SDM) -> [SDM]  "SDM（自检状态）"
  [EngineState] -> MAM/4(EngineState)
  [EngineState] -> SDM/2(S_EngineState)
  [S_SPM] -> SaveData/2(S_SPM)
  [S_CLM_Parameter] -> SaveData/3(S_ClM_Parameter)
  [MAlarm] -> SaveData/5(S_MAlarm)
  CLM/2(S_ClM_Parameter) -> [S_CLM_Parameter]  "S_CLM_Parameter（控制规律参数）"
  [S_Servo_Out] -> Bus Selector4/1
  Bus Selector4/1 -> MAM/1(S_ServoCtrlFlag)  "<ServoCtrlFlag（执行控制状态标志）>"
  [S_Servo_Out] -> SaveData/4(S_Servo_Out)
  [EngineState] -> Time Delay2/1
  [EngineState] -> FPM/2(S_EngineState)
  SaveData/15(zhenjishu) -> Bus Creator1/15  "savedata15（记录帧序号）"
  SaveData/7(EValve) -> Bus Creator1/7  "savedata7（主阀占空比）"
  SaveData/16(Tecu) -> Bus Creator1/16  "savedata16（处理器温度）"
  SaveData/20(ZhuFaShuChu) -> Bus Creator1/20  "savedata20（保留零值）"
  SaveData/21(12) -> Bus Creator1/21  "savedata21（保留零值）"
  SaveData/1(ZhiLingHuiChuan) -> Bus Creator1/1  "savedata1（指令回显）"
  SaveData/3(dianyuandianya) -> Bus Creator1/3  "savedata3（电源电压）"
  SaveData/2(T0) -> Bus Creator1/2  "savedata2（入口总温）"
  SaveData/14(GuZhangXingXi) -> Bus Creator1/14  "savedata14（故障告警）"
  SaveData/8(HuanSuanZhuanSu) -> Bus Creator1/8  "savedata8（修正转速）"
  SaveData/9(KaiGuanLiang) -> Bus Creator1/9  "savedata9（开关状态）"
  SaveData/22(BeiYong1) -> Bus Creator1/22  "savedata22（备用一）"
  SaveData/19(speed) -> Bus Creator1/19  "savedata19（飞行空速）"
  SaveData/23(BeiYong2) -> Bus Creator1/23  "savedata23（备用二）"
  SaveData/24(BeiYong3) -> Bus Creator1/24  "savedata24（备用三）"
  SaveData/12(Motor) -> Bus Creator1/12  "savedata12（电机占空比）"
  SaveData/10(WuLiZhuanSu) -> Bus Creator1/10  "savedata10（物理转速）"
  SaveData/4(T4) -> Bus Creator1/4  "savedata4（排气温度）"
  SaveData/6(Eblast) -> Bus Creator1/6  "savedata6（副阀占空比）"
  SaveData/13(FaDongJiZhuangTai) -> Bus Creator1/13  "savedata13（发动机状态）"
  SaveData/17(DianYuan) -> Bus Creator1/17  "savedata17（装订转速）"
  SaveData/5(POil) -> Bus Creator1/5  "savedata5（燃油压力）"
  SaveData/18(H) -> Bus Creator1/18  "savedata18（导航高度）"
  SaveData/11(NBump_MuBiao) -> Bus Creator1/11  "savedata11（油泵给定）"
  SaveData/25(BeiYong4) -> Bus Creator1/25  "savedata25（备用四）"
  [S_CLM_Parameter] -> ESM/1(S_CLM_Parameter)
  [EngineState] -> SaveData/1(S_EngineState)
  ControlOut/12(Out_EngineState) -> Bus Creator2/12  "EngineState（发动机状态）"
  ControlOut/1(Out_EValve_Cycle) -> Bus Creator2/1  "EValve_Cycle（主油阀周期，2毫秒/计数）"
  ControlOut/2(Out_EValve_Open) -> Bus Creator2/2  "EValve_Open（主油阀开通，2毫秒/计数）"
  ControlOut/3(Out_Eblast_Cycle) -> Bus Creator2/3  "Eblast_Cycle（副油阀周期，2毫秒/计数）"
  ControlOut/6(Out_Motor_Open) -> Bus Creator2/6, PreviousControl_上一周期控制/1  "Motor_Open（起动电机开通计数）"
  ControlOut/4(Out_Eblast_Open) -> Bus Creator2/4  "Eblast_Open（副油阀开通，2毫秒/计数）"
  ControlOut/5(Out_Motor_Cycle) -> Bus Creator2/5  "Motor_Cycle（起动电机周期计数）"
  ControlOut/7(Out_EValve_Enable) -> Bus Creator2/7  "EValve_Enable（主油阀使能）"
  ControlOut/8(Out_Eblast_Enable) -> Bus Creator2/8  "Eblast_Enable（副油阀使能）"
  ControlOut/9(Out_Motor_Enable) -> Bus Creator2/9  "Motor_Enable（起动电机使能）"
  ControlOut/10(Out_SWO_Firework) -> Bus Creator2/10  "SWO_Firework（点火器使能）"
  ControlOut/16(Out_Accelerator) -> Bus Creator2/16  "Accelerator（油泵给定控制量）"
  ControlOut/13(Out_Flag_ECUReset_Clear) -> Bus Creator2/13  "Flag_ECUReset_Clear（清除复位恢复状态）"
  ControlOut/17(Out_Nc_dem) -> Bus Creator2/17  "Nc_dem（控制目标转速）"
  ControlOut/18(Out_Nc) -> Bus Creator2/18  "Nc（反馈转速）"
  ControlOut/14(Out_Flag_ECUReset_Save) -> Bus Creator2/14  "Flag_ECUReset_Save（保存复位恢复数据）"
  ControlOut/15(Out_Flag_Reset_Enable) -> Bus Creator2/15  "Flag_Reset_Enable（软件复位请求）"
  ControlOut/11(Out_SWO_BleedAir) -> Bus Creator2/11  "SWO_BleedAir（引气阀使能）"
  [FAM] -> ControlOut/4(S_FAM)
  [S_Servo_Out] -> ControlOut/2(S_Servo_Out)
  [S_SPM] -> ControlOut/3(S_SPM)
  [EngineState] -> ControlOut/1(S_EngineState)
  [TC_IN16_T0] -> ControlRate16_二十毫秒输入/1  "T0（总温编码）"
  [TC_IN15_POil] -> ControlRate15_二十毫秒输入/1  "POil（油压原始采样）"
  [TC_IN14_BleedFeedback] -> ControlRate14_二十毫秒输入/1  "BleedFeedback（引气阀反馈）"
  [TC_IN13_ValveAlarm] -> ControlRate13_二十毫秒输入/1  "ValveAlarm（阀驱动报警）"
  [TC_IN12_AuxFeedback] -> ControlRate12_二十毫秒输入/1  "AuxFeedback（副阀反馈）"
  [TC_IN11_MainFeedback] -> ControlRate11_二十毫秒输入/1  "MainFeedback（主阀反馈）"
  [TC_IN10_FireAlarm] -> ControlRate10_二十毫秒输入/1  "FireAlarm（点火报警）"
  [TC_IN09_Tecu] -> ControlRate9_二十毫秒输入/1  "Tecu（处理器温度原始采样）"
  [TC_IN08_Power] -> ControlRate8_二十毫秒输入/1  "Power（电源电压）"
  [TC_IN07_T4] -> ControlRate7_二十毫秒输入/1  "T4（排温原始采样）"
  [TC_IN06_Nc] -> ControlRate6_二十毫秒输入/1  "Nc（反馈转速）"
  [TC_IN05_Settings] -> ControlRate5_二十毫秒输入/1  "Settings（参数装订数据）"
  [TC_IN04_ResetData] -> ControlRate4_二十毫秒输入/1  "ResetData（复位恢复数据）"
  [TC_IN03_ResetFlag] -> ControlRate3_二十毫秒输入/1  "ResetFlag（复位恢复标志）"
  [TC_IN02_Command] -> ControlRate2_二十毫秒输入/1  "Command（上位机指令数据）"
  [TC_IN01_RxFlag] -> ControlRate1_二十毫秒输入/1  "RxFlag（新指令标志）"
  Bus Creator1/1 -> savedata/1, [TC_BUS_SaveData]  "SaveData（运行记录总线）"
  Bus Creator2/1 -> Controldata/1, [TC_BUS_ControlData]  "ControlData（执行控制总线）"
  ControlRate1_二十毫秒输入/1 -> COMMRead_ISM/1(S_Flag_rx_suc)
  ControlRate2_二十毫秒输入/1 -> COMMRead_ISM/2(S_PF_MyUsart2_Rxdata)
  ControlRate3_二十毫秒输入/1 -> COMMRead_ISM/3(S_Flag_ECUReset)
  ControlRate4_二十毫秒输入/1 -> COMMRead_ISM/4(S_ECUReset_Information)
  ControlRate5_二十毫秒输入/1 -> COMMRead_ISM/5(S_MySet_Rxdata)
  ControlRate6_二十毫秒输入/1 -> COMMRead_ISM/6(S_Nc)
  ControlRate7_二十毫秒输入/1 -> COMMRead_ISM/7(S_T4)
  ControlRate8_二十毫秒输入/1 -> COMMRead_ISM/8(S_Vpower)
  ControlRate9_二十毫秒输入/1 -> COMMRead_ISM/9(S_Tecu)
  ControlRate10_二十毫秒输入/1 -> COMMRead_ISM/10(S_SWI_Firework)
  ControlRate11_二十毫秒输入/1 -> COMMRead_ISM/11(S_SWI_EValve)
  ControlRate12_二十毫秒输入/1 -> COMMRead_ISM/12(S_SWI_Eblast)
  ControlRate13_二十毫秒输入/1 -> COMMRead_ISM/13(S_SWI_ValveErr)
  ControlRate14_二十毫秒输入/1 -> COMMRead_ISM/15(S_SWI_BleedAir)
  ControlRate15_二十毫秒输入/1 -> COMMRead_ISM/16(S_POil)
  ControlRate16_二十毫秒输入/1 -> COMMRead_ISM/17(S_T0)
  PreviousControl_上一周期控制/1 -> [TC_IO_PreviousMotor]  "PreviousMotor（上一周期电机开通量）"
  Time Delay2/1 -> COMMRead_ISM/14(S_EngineState)
  COMMRead_ISM/1(S_SPM) -> [S_SPM], ESM/2(S_SPM), FPM/1(S_SPM), SDM/1(S_SPM), MAM/3(S_SPM), CLM/1(S_SPM)  "S_SPM（输入综合信息）"
  LogPack_运行记录列定义/1(LogVector（二十七项记录）) -> SDLog_官方SD卡记录/1
  LogTime_记录时钟/1 -> LogPack_运行记录列定义/2(Time（时间秒）)  "Log_Time（记录时间秒）"
  [TC_BUS_SaveData] -> LogPack_运行记录列定义/1(Savedata（运行数据总线）)  "SaveData（运行记录总线）"
  FRAM_复位恢复事务/9(Errors（写后验证失败次数）) -> LogErrors_恢复错误记录/1
  FRAM_复位恢复事务/8(Info20（二十字节恢复内容）) -> [TC_IO_RecoveryData]
  FRAM_复位恢复事务/7(Restore（一次恢复通知）) -> [TC_IO_RecoveryFlag]
  FRAM_复位恢复事务/6(En1（写使能发送允许）) -> FRAM_写使能命令/Enable
  FRAM_复位恢复事务/5(Tx1（写使能命令）) -> FRAM_写使能命令/1(In1)
  FRAM_复位恢复事务/4(En4（提交帧发送允许）) -> FRAM_四字节提交/Enable
  FRAM_复位恢复事务/3(Tx4（失效或提交帧）) -> FRAM_四字节提交/1(In1)
  FRAM_复位恢复事务/2(En67（完整帧发送允许）) -> FRAM_Read_读取恢复/Enable
  FRAM_复位恢复事务/1(Tx67（完整读写帧）) -> FRAM_Read_读取恢复/1(In1)
  FRAM_RxDelay_传输反馈/1 -> FRAM_复位恢复事务/4(Rx67（上一周期FRAM返回帧）)  "FRAM_LastReceived（上一毫秒返回帧）"
  FRAM_DataDelay_记录快照/1 -> FRAM_复位恢复事务/3(Data（运行数据总线）)
  FRAM_SendDelay_协议快照/1 -> FRAM_复位恢复事务/2(Send（通信回传总线）)
  FRAM_ControlDelay_控制快照/1 -> FRAM_复位恢复事务/1(Control（执行控制总线）)
  FRAM_Read_读取恢复/1(Out1) -> FRAM_RxDelay_传输反馈/1  "FRAM_Received（存储器返回数据）"
  FRAM_写使能命令/1(Out1) -> FRAM_使能返回终止/1
  FRAM_四字节提交/1(Out1) -> FRAM_提交返回终止/1
  [TC_BUS_SendData] -> FRAM_SendDelay_协议快照/1  "SendData（通信命令总线）"
  [TC_BUS_ControlData] -> FRAM_ControlDelay_控制快照/1  "ControlData（执行控制总线）"
  [TC_BUS_SaveData] -> FRAM_DataDelay_记录快照/1  "SaveData（运行记录总线）"
  LogErrors_恢复错误记录/1 -> LogPack_运行记录列定义/3(Errors（恢复错误次数）)  "Log_Errors（记录恢复错误次数）"
  Clock_模型时钟/1 -> [TC_IO_ModelTime], LogTime_记录时钟/1, FRAM_复位恢复事务/5(Seconds（当前时间秒）)  "ModelTime（模型时间秒）"
  BoardOutput_串口封装与阀门时序/8(Length2（油泵发送长度）) -> USART2_发送协议帧/2
  BoardOutput_串口封装与阀门时序/7(Tx2（油泵指令帧）) -> USART2_发送协议帧/1
  BoardOutput_串口封装与阀门时序/6(Length1（电机发送长度）) -> USART1_发送协议帧/2
  BoardOutput_串口封装与阀门时序/5(Tx1（电机指令帧）) -> USART1_发送协议帧/1
  BoardOutput_串口封装与阀门时序/4(Length4（回传发送长度）) -> UART4_发送协议帧/2
  BoardOutput_串口封装与阀门时序/3(Tx4（上位机回传帧）) -> UART4_发送协议帧/1
  BoardOutput_串口封装与阀门时序/2(PortD（D口三路电平）) -> GPIOD_使能镜像点火/1
  BoardOutput_串口封装与阀门时序/1(PortE（E口三路电平）) -> GPIOE_阀驱动输出/1
  [TC_IO_ModelTime] -> BoardOutput_串口封装与阀门时序/5(Seconds（当前秒数）)  "ModelTime（模型时间秒）"
  [TC_BUS_SendData] -> BoardOutput_串口封装与阀门时序/2(Send（回传及外设命令总线）)  "SendData（通信命令总线）"
  [TC_BUS_ControlData] -> BoardOutput_串口封装与阀门时序/1(Control（执行控制总线）)  "ControlData（执行控制总线）"
  SendData/22(rt) -> Bus Creator3/22  "senddata22（帧序号占位）"
  Bus Creator3/1 -> [TC_BUS_SendData], senddata/1  "SendData（通信命令总线）"
  [S_SPM] -> SendData/1(S_SPM)
  [SDM] -> SendData/2(S_SDM)
  [S_Servo_Out] -> SendData/3(S_Servo_Out)
  [EngineState] -> SendData/4(S_EngineState)
  [MAlarm] -> SendData/5(S_MAlarm)
  SendData/3(ZhiLingHuiChuan) -> Bus Creator3/3  "senddata3（指令回显）"
  SendData/4(T0) -> Bus Creator3/4  "senddata4（总温编码）"
  SendData/5(dianyuandianya) -> Bus Creator3/5  "senddata5（电压编码）"
  SendData/6(T4_H) -> Bus Creator3/6  "senddata6（排温高字节）"
  SendData/7(T4_L) -> Bus Creator3/7  "senddata7（排温低字节）"
  SendData/8(POil_H) -> Bus Creator3/8  "senddata8（油压高字节）"
  SendData/9(POil_L) -> Bus Creator3/9  "senddata9（油压低字节）"
  SendData/10(Eblast) -> Bus Creator3/10  "senddata10（副阀占空比）"
  SendData/11(EValve) -> Bus Creator3/11  "senddata11（主阀占空比）"
  SendData/12(HuanSuanZhuanSuH) -> Bus Creator3/12  "senddata12（修正转速高）"
  SendData/13(HuanSuanZhuanSuL) -> Bus Creator3/13  "senddata13（修正转速低）"
  SendData/14(KaiGuanLiang) -> Bus Creator3/14  "senddata14（开关状态）"
  SendData/15(WuLiZhuanSuH1) -> Bus Creator3/15  "senddata15（物理转速高）"
  SendData/16(WuLiZhuanSuL1) -> Bus Creator3/16  "senddata16（物理转速低）"
  SendData/17(NBump_MuBiaoH) -> Bus Creator3/17  "senddata17（油泵给定高）"
  SendData/18(NBump_MuBiaoL) -> Bus Creator3/18  "senddata18（油泵给定低）"
  SendData/19(Motor) -> Bus Creator3/19  "senddata19（电机命令）"
  SendData/20(FaDongJiZhuangTai) -> Bus Creator3/20  "senddata20（发动机状态）"
  SendData/21(GuZhangXingXi) -> Bus Creator3/21  "senddata21（故障告警）"
  SendData/23(TECU) -> Bus Creator3/23  "senddata23（处理器温度码）"
  SendData/24(MuBiaoiZhuanSuH2) -> Bus Creator3/24  "senddata24（目标转速高）"
  SendData/1(ChuanShuBiaoZhi) -> Bus Creator3/1  "senddata1（发送允许）"
  SendData/2(ShuJuChangDu) -> Bus Creator3/2  "senddata2（载荷字节数）"
  SendData/25(MuBiaoZhuanSuL2) -> Bus Creator3/25  "senddata25（目标转速低）"
  SendData/29(NBumpL) -> Bus Creator3/29  "senddata29（装订转速低）"
  SendData/28(NBumpH) -> Bus Creator3/28  "senddata28（装订转速高）"
  SendData/26(QW) -> Bus Creator3/26  "senddata26（实测泵速高占位）"
  SendData/27(ER) -> Bus Creator3/27  "senddata27（实测泵速低占位）"
  GPIOE_PE15_Feedback/1 -> GPIOE_FeedbackVector/3
  GPIOE_PE14_Feedback/1 -> GPIOE_FeedbackVector/2
  GPIOE_PE13_Feedback/1 -> GPIOE_FeedbackVector/1  "Valve_Feedback（引气、主阀、副阀反馈）"
  GPIOD_AlarmVector/1 -> BoardInput_输入换算与协议解析/9(GPIOD（D口两路反馈）)
  GPIOD_PD9_Alarm/1 -> GPIOD_AlarmVector/2
  GPIOD_PD8_Alarm/1 -> GPIOD_AlarmVector/1  "Alarm_Input（阀与点火报警）"
  BoardInput_输入换算与协议解析/16(T0（总温编码）) -> [TC_IN16_T0]
  BoardInput_输入换算与协议解析/15(POil（油压原始计数）) -> [TC_IN15_POil]
  BoardInput_输入换算与协议解析/14(Bleed（放气反馈）) -> [TC_IN14_BleedFeedback]
  BoardInput_输入换算与协议解析/13(Valve（阀使能反馈）) -> [TC_IN13_ValveAlarm]
  BoardInput_输入换算与协议解析/12(Aux（副阀反馈）) -> [TC_IN12_AuxFeedback]
  BoardInput_输入换算与协议解析/11(Main（主阀反馈）) -> [TC_IN11_MainFeedback]
  BoardInput_输入换算与协议解析/10(Fire（点火反馈）) -> [TC_IN10_FireAlarm]
  BoardInput_输入换算与协议解析/9(TECU（处理器温度原始计数）) -> [TC_IN09_Tecu]
  BoardInput_输入换算与协议解析/8(Power（电源电压）) -> [TC_IN08_Power]
  BoardInput_输入换算与协议解析/7(T4（排温原始计数）) -> [TC_IN07_T4]
  BoardInput_输入换算与协议解析/6(Speed（控制用转速）) -> [TC_IN06_Nc]
  BoardInput_输入换算与协议解析/5(Setting（预留装订数据）) -> [TC_IN05_Settings]
  BoardInput_输入换算与协议解析/4(ResetInfo（恢复内容）) -> [TC_IN04_ResetData]
  [TC_IO_ModelTime] -> BoardInput_输入换算与协议解析/15(Seconds（当前秒数）)  "ModelTime（模型时间秒）"
  [TC_IO_RecoveryData] -> BoardInput_输入换算与协议解析/14(FRAMInfo（复位恢复内容）)  "RecoveryData（恢复数据）"
  [TC_IO_RecoveryFlag] -> BoardInput_输入换算与协议解析/13(FRAMFlag（复位恢复通知）)  "RecoveryFlag（恢复有效标志）"
  [TC_IO_PreviousMotor] -> BoardInput_输入换算与协议解析/12(PreviousMotor（上一周期电机给定）)  "PreviousMotor（上一周期电机开通量）"
  TIM3_转速边沿捕获/2 -> BoardInput_输入换算与协议解析/11(CountCapture（有效捕获个数）)  "Capture_Count（有效边沿数）"
  TIM3_转速边沿捕获/1 -> BoardInput_输入换算与协议解析/10(Capture（转速捕获计数）)  "Capture_Ticks（转速边沿计数）"
  USART2_接收字节流/1 -> BoardOutput_串口封装与阀门时序/3(PumpRx（油泵反馈字节）), BoardInput_输入换算与协议解析/6(Rx2（油泵接收字节）)  "Pump_Bytes（油泵反馈字节流）"
  USART2_接收字节流/2 -> BoardOutput_串口封装与阀门时序/4(PumpCount（油泵有效字节数）), BoardInput_输入换算与协议解析/7(Count2（油泵有效字节数）)  "Pump_Length（油泵有效字节数）"
  ADC1_八路采样/1 -> BoardInput_输入换算与协议解析/1(ADC（八路模拟采样）)  "ADC_Raw（八路原始采样）"
  UART4_接收字节流/1 -> BoardInput_输入换算与协议解析/2(Rx4（上位机接收字节）)  "Command_Bytes（上位机字节流）"
  UART4_接收字节流/2 -> BoardInput_输入换算与协议解析/3(Count4（上位机有效字节数）)  "Command_Length（上位机有效字节数）"
  USART1_接收字节流/1 -> BoardInput_输入换算与协议解析/4(Rx1（电机接收字节）)  "Motor_Bytes（电机反馈字节流）"
  USART1_接收字节流/2 -> BoardInput_输入换算与协议解析/5(Count1（电机有效字节数）)  "Motor_Length（电机有效字节数）"
  BoardInput_输入换算与协议解析/1(Flag（新命令通知）) -> [TC_IN01_RxFlag]
  BoardInput_输入换算与协议解析/2(Command（最近有效命令）) -> [TC_IN02_Command]
  BoardInput_输入换算与协议解析/3(ResetFlag（恢复通知）) -> [TC_IN03_ResetFlag]
  GPIOE_FeedbackVector/1 -> BoardInput_输入换算与协议解析/8(GPIOE（E口三路反馈）)
